simulink model "youBot_Arm"  (R2025a)
settings: Solver=ode15s  StartTime=0.0  StopTime=20  MaxStep=1e-2  RelTol=1e-3  AbsTol=1e-4
model workspace: external: MATLAB File youBot_DataFile.m (data not in the file)
undefined symbols (not defined in the file): Extr_Data_LinkHoles, Qt, sigbuilder_block, smiData, X, Y, YBT_Par, Z
libraries: sm_lib x193, nesl_utility x130, fl_lib x53, simulink x13, Parts_Lib x10, MyMath_lib x8, Motor_Lib x5, Contact_Forces_Lib x4, ee_lib x2, sdl_lib x2
(part 4 of 8)

== system youBot_Arm/Arm/Wrist/Wrist_1_RIGID ==
  ReferenceFrame : sm_lib/Frames and Transforms/Reference Frame
  Solid : sm_lib/Body Elements/File Solid  ExtGeomFileName=Wrist.step  UnitType=FromFile  ExtGeomFileUnits=m  StepReaderType=HEX  ExportConvexHullGeometry=off  InertiaType=Custom  BasedOnType=Density  Density=1000  DensityUnits=kg/m^3  Mass=smiData.Solid(9).mass  MassUnits=kg  CenterOfMass=smiData.Solid(9).CoM  CenterOfMassUnits=m  MomentsOfInertia=smiData.Solid(9).MoI  MomentsOfInertiaUnits=kg*m^2  ProductsOfInertia=smiData.Solid(9).PoI  ProductsOfInertiaUnits=kg*m^2  GraphicType=FromGeometry  MarkerShape=Sphere  MarkerSize=10  GraphicVisPropType=SimpleVisualProperties  GraphicDiffuseColor=smiData.Solid(9).color  GraphicOpacity=smiData.Solid(9).opacity  GraphicSpecularColor=[0.5 0.5 0.5 1.0]  GraphicAmbientColor=[0.15 0.15 0.15 1.0]  GraphicEmissiveColor=[0.0 0.0 0.0 1.0]  GraphicShininess=75  DoExposeReferenceFrame=on  SerializedFrames=<Frames/>
  Transform : sm_lib/Frames and Transforms/Rigid Transform  RotationMethod=ArbitraryAxis  FollAlignAxisA=+X  BaseAlignAxisA=+Y  FollAlignAxisB=+Y  BaseAlignAxisB=+Z  RotationStandardAxis=+Z  RotationAngle=smiData.RigidTransform(27).angle  RotationAngleUnits=rad  RotationArbitraryAxis=smiData.RigidTransform(27).axis  RotationSequenceAxes=FollowerAxes  RotationSequence=XYX  RotationSequenceAngles=[0 0 0]  RotationSequenceAnglesUnits=deg  RotationMatrix=[1 0 0; 0 1 0; 0 0 1]  Quaternion=[1 0 0 0]  TranslationMethod=Cartesian  TranslationCartesianOffset=smiData.RigidTransform(27).translation  TranslationCartesianOffsetUnits=m  TranslationStandardAxis=+Z  TranslationStandardOffset=0  TranslationStandardOffsetUnits=m  TranslationROffset=0  TranslationROffsetUnits=m  TranslationThetaOffset=0  TranslationThetaOffsetUnits=deg  TranslationZOffset=0  TranslationZOffsetUnits=m
  Transform1 : sm_lib/Frames and Transforms/Rigid Transform  RotationMethod=ArbitraryAxis  FollAlignAxisA=+X  BaseAlignAxisA=+Y  FollAlignAxisB=+Y  BaseAlignAxisB=+Z  RotationStandardAxis=+Z  RotationAngle=smiData.RigidTransform(30).angle  RotationAngleUnits=rad  RotationArbitraryAxis=smiData.RigidTransform(30).axis  RotationSequenceAxes=FollowerAxes  RotationSequence=XYX  RotationSequenceAngles=[0 0 0]  RotationSequenceAnglesUnits=deg  RotationMatrix=[1 0 0; 0 1 0; 0 0 1]  Quaternion=[1 0 0 0]  TranslationMethod=Cartesian  TranslationCartesianOffset=smiData.RigidTransform(30).translation  TranslationCartesianOffsetUnits=m  TranslationStandardAxis=+Z  TranslationStandardOffset=0  TranslationStandardOffsetUnits=m  TranslationROffset=0  TranslationROffsetUnits=m  TranslationThetaOffset=0  TranslationThetaOffsetUnits=deg  TranslationZOffset=0  TranslationZOffsetUnits=m
  F1 : PMIOPort  Side=Left
  F : PMIOPort  Port=2  Side=Right
  connections:
  Solid/RConn1 -- ReferenceFrame/RConn1 -- Transform/LConn1 -- Transform1/LConn1
  Transform/RConn1 -- F/RConn1
  Transform1/RConn1 -- F1/RConn1

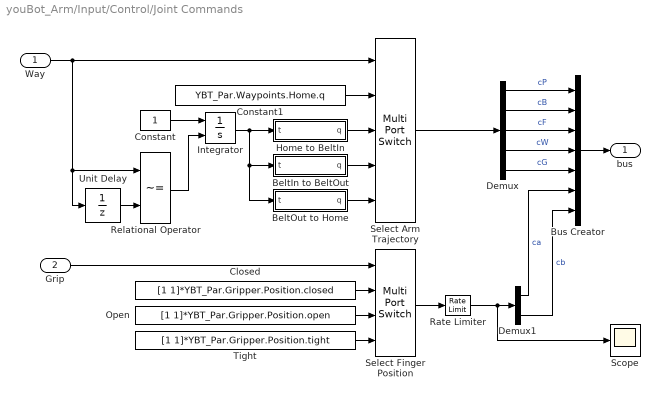
== system youBot_Arm/Input/Control/Joint Commands ==
  Way : Inport
  Grip : Inport  Port=2
  BeltIn to BeltOut : Subsystem
  BeltOut to Home : Subsystem
  Bus Creator : BusCreator  Inputs=7
  Closed : Constant  Value=[1 1]*YBT_Par.Gripper.Position.closed
  Constant : Constant  SampleTime=0
  Constant1 : Constant  Value=YBT_Par.Waypoints.Home.q
  Demux : Demux  Outputs=5
  Demux1 : Demux  Outputs=2
  Home to BeltIn : Subsystem
  Integrator : Integrator  ExternalReset=rising
  Open : Constant  Value=[1 1]*YBT_Par.Gripper.Position.open
  Rate Limiter : RateLimiter  RisingSlewLimit=YBT_Par.Finger_A.Motor.max_spd  FallingSlewLimit=-YBT_Par.Finger_A.Motor.max_spd  SampleTimeMode=inherited
  Relational Operator : RelationalOperator  Operator=~=  OutDataTypeStr=boolean  RndMeth=Simplest  InputSameDT=off
  Scope : Scope
      settings: ActiveDisplayYMinimum=-4.375  ActiveDisplayYMaximum=39.375
  Select Arm Trajectory : MultiPortSwitch  DataPortOrder=Zero-based contiguous  Inputs=4  zeroidx=on  SaturateOnIntegerOverflow=off  InputSameDT=off
  Select Finger Position : MultiPortSwitch  DataPortOrder=Zero-based contiguous  zeroidx=on  SaturateOnIntegerOverflow=off  InputSameDT=off
  Tight : Constant  Value=[1 1]*YBT_Par.Gripper.Position.tight
  Unit Delay : UnitDelay  SampleTime=1e-2  HasFrameUpgradeWarning=on
  bus : Outport  VectorParamsAs1DForOutWhenUnconnected=off
  wires:
  Bus Creator/1 -> bus/1
  Demux/5 -> Bus Creator/5  "cG"
  Demux/4 -> Bus Creator/4  "cW"
  Demux/3 -> Bus Creator/3  "cF"
  Demux/2 -> Bus Creator/2  "cB"
  Demux1/2 -> Bus Creator/7  "cb"
  Demux1/1 -> Bus Creator/6  "ca"
  Select Finger Position/1 -> Rate Limiter/1
  Grip/1 -> Select Finger Position/1
  Tight/1 -> Select Finger Position/4
  Open/1 -> Select Finger Position/3
  Closed/1 -> Select Finger Position/2
  Demux/1 -> Bus Creator/1  "cP"
  Integrator/1 -> BeltOut to Home/1(t), BeltIn to BeltOut/1(t), Home to BeltIn/1(t)
  Constant1/1 -> Select Arm Trajectory/2
  Relational Operator/1 -> Integrator/2
  Select Arm Trajectory/1 -> Demux/1
  Home to BeltIn/1(q) -> Select Arm Trajectory/3
  BeltIn to BeltOut/1(q) -> Select Arm Trajectory/4
  Unit Delay/1 -> Relational Operator/2
  Constant/1 -> Integrator/1
  Way/1 -> Select Arm Trajectory/1, Relational Operator/1, Unit Delay/1
  BeltOut to Home/1(q) -> Select Arm Trajectory/5
  Rate Limiter/1 -> Scope/1, Demux1/1

== system youBot_Arm/Input/Control/Logging ==
  S : Inport
  Bus Selector1 : BusSelector  Commented=on  OutputSignals=BeltIn.Box,BeltIn.LC,BeltOut.Box,BeltOut.LC
  Bus Selector2 : BusSelector  Commented=on  OutputSignals=Belts
  From Workspace : FromWorkspace  Commented=on  VariableName=chartInputs  OutDataTypeStr=Bus: Belts
  Scope : Scope  Commented=on  NumInputPorts=4
      settings: ActiveDisplayYMinimum=-0.125  ActiveDisplayYMaximum=1.125
  To Workspace : ToWorkspace  Commented=on  VariableName=chartInputs  SaveFormat=Timeseries  SampleTime=0.1
  wires:
  From Workspace/1 -> Bus Selector1/1
  Bus Selector1/2 -> Scope/2  "<LC>"
  Bus Selector1/3 -> Scope/3  "<Box>"
  Bus Selector1/4 -> Scope/4  "<LC>"
  Bus Selector1/1 -> Scope/1  "<Box>"
  Bus Selector2/1 -> To Workspace/1  "<Belts>"
  S/1 -> Bus Selector2/1

== system youBot_Arm/Input/Control Belt/Control Belt In ==
  BeltOut : Inport
  Sensor : Inport  Port=2
  Product : Product
  Scope : Scope  NumInputPorts=3
      settings: ActiveDisplayYMinimum=-0.125  ActiveDisplayYMaximum=1.125
  On : Outport  VectorParamsAs1DForOutWhenUnconnected=off
  wires:
  Sensor/1 -> Scope/3, Product/2
  Product/1 -> Scope/1, On/1  "vx"
  BeltOut/1 -> Scope/2, Product/1

== system youBot_Arm/Input/Control Belt/Control Belt Out ==
  BeltOut : Inport
  Sensor : Inport  Port=2
  Product : Product
  Scope : Scope  NumInputPorts=3
      settings: ActiveDisplayYMinimum=-0.125  ActiveDisplayYMaximum=1.125
  On : Outport  VectorParamsAs1DForOutWhenUnconnected=off
  wires:
  BeltOut/1 -> Product/1, Scope/2
  Product/1 -> On/1, Scope/1  "vx"
  Sensor/1 -> Product/2, Scope/3

== system youBot_Arm/Input/Control Belt/Robot Commands ==
  Bus Creator : BusCreator  Tag=Bus Creator  Inputs=7
  FromWs : FromWorkspace  Tag=STV FromWs  VariableName=tuvar
      SigBuilderData=|
      | common.afterFinalStr = 'Extrapolate'
      | common.sampleTime = 0
      | dataSet(1).timeRange = [0 10]
      | dataSet(1).name = 'All 35'
      | dataSet(2).timeRange = [0 20]
      | dataSet(2).name = 'Box 40 cm'
      | dataSet(3).timeRange = [0 20]
      | dataSet(3).name = 'Box 40 cm Flip'
      | dataSet(4).timeRange = [0 20]
      | dataSet(4).name = 'Box 40 cm upDown'
      | dataSet(5).timeRange = [0 3]
      | dataSet(5).name = 'Opt Flip Orig'
      | dataSet(6).timeRange = [0 4]
      | dataSet(6).name = 'Opt Flip Test'
      | dataSet(7).timeRange = [0 14]
      | dataSet(7).name = 'Test Pivot'
      | dataSet(8).timeRange = [0 14]
      | dataSet(8).name = 'Test Bicep'
      | dataSet(9).timeRange = [0 14]
      | dataSet(9).name = 'Test Forearm'
      | dataSet(10).timeRange = [0 14]
      | dataSet(10).name = 'Test Wrist'
      | sbobj.Groups(1).Name = 'All 35'
      | sbobj.Groups(1).Signals(1).Name = 'cP'
      | sbobj.Groups(1).Signals(1).XData = [0 2 4 6 8 10]
      | sbobj.Groups(1).Signals(1).YData = [0 0 35 35 0 0]
      | sbobj.Groups(1).Signals(2).Name = 'cB'
      | sbobj.Groups(1).Signals(2).XData = [0 2 4 6 8 10]
      | sbobj.Groups(1).Signals(2).YData = [0 0 35 35 0 0]
      | sbobj.Groups(1).Signals(3).Name = 'cF'
      | sbobj.Groups(1).Signals(3).XData = [0 2 4 6 8 10]
      | sbobj.Groups(1).Signals(3).YData = [0 0 35 35 0 0]
      | sbobj.Groups(1).Signals(4).Name = 'cW'
      | sbobj.Groups(1).Signals(4).XData = [0 2 4 6 8 10]
      | sbobj.Groups(1).Signals(4).YData = [0 0 35 35 0 0]
      | sbobj.Groups(1).Signals(5).Name = 'cG'
      | sbobj.Groups(1).Signals(5).XData = [0 2 4 6 8 10]
      | sbobj.Groups(1).Signals(5).YData = [0 0 35 35 0 0]
      | sbobj.Groups(1).Signals(6).Name = 'ca'
      | sbobj.Groups(1).Signals(6).XData = [0 2 4 6 8 10]
      | sbobj.Groups(1).Signals(6).YData = [0 0 35 35 0 0]
      | sbobj.Groups(1).Signals(7).Name = 'cb'
      | sbobj.Groups(1).Signals(7).XData = [0 2 4 6 8 10]
      | sbobj.Groups(1).Signals(7).YData = [0 0 35 35 0 0]
      | sbobj.Groups(2).Name = 'Box 40 cm'
      | sbobj.Groups(2).Signals(1).Name = 'cP'
      | sbobj.Groups(2).Signals(1).XData = [0 2 4 5.5 7 9 14 18 20]
      | sbobj.Groups(2).Signals(1).YData = [0 0 0 0 0 -90 -90 0 0]
      | sbobj.Groups(2).Signals(2).Name = 'cB'
      | sbobj.Groups(2).Signals(2).XData = [0 2 4 6 7 8 10 13 18 20]
      | sbobj.Groups(2).Signals(2).YData = [0 0 60 60 50 50 59 59 0 0]
      | sbobj.Groups(2).Signals(3).Name = 'cF'
      | sbobj.Groups(2).Signals(3).XData = [0 2 3 14 18 20]
      | sbobj.Groups(2).Signals(3).YData = [0 0 115 115 0 0]
      | sbobj.Groups(2).Signals(4).Name = 'cW'
      | sbobj.Groups(2).Signals(4).XData = [0 2 4 14 18 20]
      | sbobj.Groups(2).Signals(4).YData = [0 0 -85 -85 0 0]
      | sbobj.Groups(2).Signals(5).Name = 'cG'
      | sbobj.Groups(2).Signals(5).XData = [0 2 4 6 8 20]
      | sbobj.Groups(2).Signals(5).YData = [0 0 0 0 0 0]
      | sbobj.Groups(2).Signals(6).Name = 'ca'
      | sbobj.Groups(2).Signals(6).XData = [0 2 3 4.5 5 12 12.2 20]
      | sbobj.Groups(2).Signals(6).YData = [0 0 35 35 29 29 31 31]
      | sbobj.Groups(2).Signals(7).Name = 'cb'
      | sbobj.Groups(2).Signals(7).XData = [0 2 3 4.5 5 12 12.2 20]
      | sbobj.Groups(2).Signals(7).YData = [0 0 35 35 29 29 31 31]
      | sbobj.Groups(2).TimeRange = [0 20]
      | sbobj.Groups(3).Name = 'Box 40 cm Flip'
      | sbobj.Groups(3).Signals(1).Name = 'cP'
      | sbobj.Groups(3).Signals(1).XData = [0 2 4 5.5 6 10 16 18 20]
      | sbobj.Groups(3).Signals(1).YData = [0 0 0 0 0 90 90 0 0]
      | sbobj.Groups(3).Signals(2).Name = 'cB'
      | sbobj.Groups(3).Signals(2).XData = [0 2 4 5.5 10 14 18 20]
      | sbobj.Groups(3).Signals(2).YData = [0 0 60 60 -60 -60 0 0]
      | sbobj.Groups(3).Signals(3).Name = 'cF'
      | sbobj.Groups(3).Signals(3).XData = [0 2 3.5 5.5 10 14 18 20]
      | sbobj.Groups(3).Signals(3).YData = [0 0 115 115 -110 -110 0 0]
      | sbobj.Groups(3).Signals(4).Name = 'cW'
      | sbobj.Groups(3).Signals(4).XData = [0 2 3.5 5.5 10 14 18 20]
      | sbobj.Groups(3).Signals(4).YData = [0 0 -85 -85 79 79 0 0]
      | sbobj.Groups(3).Signals(5).Name = 'cG'
      | sbobj.Groups(3).Signals(5).XData = [0 2 4 6 8 20]
      | sbobj.Groups(3).Signals(5).YData = [0 0 0 0 0 0]
      | sbobj.Groups(3).Signals(6).Name = 'ca'
      | sbobj.Groups(3).Signals(6).XData = [0 2 2.5 4.5 5 11.5 12 20]
      | sbobj.Groups(3).Signals(6).YData = [0 0 35 35 29 29 31 31]
      | sbobj.Groups(3).Signals(7).Name = 'cb'
      | sbobj.Groups(3).Signals(7).XData = [0 2 2.5 4.5 5 11.5 12 20]
      | sbobj.Groups(3).Signals(7).YData = [0 0 35 35 29 29 31 31]
      | sbobj.Groups(3).TimeRange = [0 20]
      | sbobj.Groups(4).Name = 'Box 40 cm upDown'
      | sbobj.Groups(4).Signals(1).Name = 'cP'
      | sbobj.Groups(4).Signals(1).XData = [0 2 4 5.5 7 9 14 18 20]
      | sbobj.Groups(4).Signals(1).YData = [0 0 0 0 0 360 360 0 0]
      | sbobj.Groups(4).Signals(2).Name = 'cB'
      | sbobj.Groups(4).Signals(2).XData = [0 2 4 6 7 8 10 13 18 20]
      | sbobj.Groups(4).Signals(2).YData = [0 0 60 60 50 50 59 59 0 0]
      | sbobj.Groups(4).Signals(3).Name = 'cF'
      | sbobj.Groups(4).Signals(3).XData = [0 2 3 14 18 20]
      | sbobj.Groups(4).Signals(3).YData = [0 0 115 115 0 0]
      | sbobj.Groups(4).Signals(4).Name = 'cW'
      | sbobj.Groups(4).Signals(4).XData = [0 2 4 14 18 20]
      | sbobj.Groups(4).Signals(4).YData = [0 0 -85 -85 0 0]
      | sbobj.Groups(4).Signals(5).Name = 'cG'
      | sbobj.Groups(4).Signals(5).XData = [0 2 4 6 8 20]
      | sbobj.Groups(4).Signals(5).YData = [0 0 0 0 0 0]
      | sbobj.Groups(4).Signals(6).Name = 'ca'
      | sbobj.Groups(4).Signals(6).XData = [0 2 3 4.5 5 12 12.2 20]
      | sbobj.Groups(4).Signals(6).YData = [0 0 35 35 29 29 31 31]
      | sbobj.Groups(4).Signals(7).Name = 'cb'
      | sbobj.Groups(4).Signals(7).XData = [0 2 3 4.5 5 12 12.2 20]
      | sbobj.Groups(4).Signals(7).YData = [0 0 35 35 29 29 31 31]
      | sbobj.Groups(4).TimeRange = [0 20]
      | sbobj.Groups(5).Name = 'Opt Flip Orig'
      | sbobj.Groups(5).Signals(1).Name = 'cP'
      | sbobj.Groups(5).Signals(1).XData = [0 3]
      | sbobj.Groups(5).Signals(1).YData = [0 90]
      | sbobj.Groups(5).Signals(2).Name = 'cB'
      | sbobj.Groups(5).Signals(2).XData = [0 3]
      | sbobj.Groups(5).Signals(2).YData = [60 -60]
      | sbobj.Groups(5).Signals(3).Name = 'cF'
      | sbobj.Groups(5).Signals(3).XData = [0 3]
      | sbobj.Groups(5).Signals(3).YData = [115 -110]
      | sbobj.Groups(5).Signals(4).Name = 'cW'
      | sbobj.Groups(5).Signals(4).XData = [0 3]
      | sbobj.Groups(5).Signals(4).YData = [-85 79]
      | sbobj.Groups(5).Signals(5).Name = 'cG'
      | sbobj.Groups(5).Signals(5).XData = [0 2 3]
      | sbobj.Groups(5).Signals(5).YData = [0 0 0]
      | sbobj.Groups(5).Signals(6).Name = 'ca'
      | sbobj.Groups(5).Signals(6).XData = [0 3]
      | sbobj.Groups(5).Signals(6).YData = [0 0]
      | sbobj.Groups(5).Signals(7).Name = 'cb'
      | sbobj.Groups(5).Signals(7).XData = [0 3]
      | sbobj.Groups(5).Signals(7).YData = [0 0]
      | sbobj.Groups(5).TimeRange = [0 3]
      | sbobj.Groups(6).Name = 'Opt Flip Test'
      | sbobj.Groups(6).Signals(1).Name = 'cP'
      | sbobj.Groups(6).Signals(1).XData = [0 3 4]
      | sbobj.Groups(6).Signals(1).YData = [0 90 90]
      | sbobj.Groups(6).Signals(2).Name = 'cB'
      | sbobj.Groups(6).Signals(2).XData = [0 3 4]
      | sbobj.Groups(6).Signals(2).YData = [60 -60 -60]
      | sbobj.Groups(6).Signals(3).Name = 'cF'
      | sbobj.Groups(6).Signals(3).XData = [0 3 4]
      | sbobj.Groups(6).Signals(3).YData = [115 -110 -110]
      | sbobj.Groups(6).Signals(4).Name = 'cW'
      | sbobj.Groups(6).Signals(4).XData = [0 3 4]
      | sbobj.Groups(6).Signals(4).YData = [-85 79 79]
      | sbobj.Groups(6).Signals(5).Name = 'cG'
      | sbobj.Groups(6).Signals(5).XData = [0 2 4]
      | sbobj.Groups(6).Signals(5).YData = [0 0 0]
      | sbobj.Groups(6).Signals(6).Name = 'ca'
      | sbobj.Groups(6).Signals(6).XData = [0 4]
      | sbobj.Groups(6).Signals(6).YData = [0 0]
      | sbobj.Groups(6).Signals(7).Name = 'cb'
      | sbobj.Groups(6).Signals(7).XData = [0 4]
      | sbobj.Groups(6).Signals(7).YData = [0 0]
      | sbobj.Groups(6).TimeRange = [0 4]
      | sbobj.Groups(7).Name = 'Test Pivot'
      | sbobj.Groups(7).Signals(1).Name = 'cP'
      | sbobj.Groups(7).Signals(1).XData = [0 2 4 5 8.8 10 12 14]
      | sbobj.Groups(7).Signals(1).YData = [0 0 -169 -169 169 169 0 0]
      | sbobj.Groups(7).Signals(2).Name = 'cB'
      | sbobj.Groups(7).Signals(2).XData = [0 2 3 5 6.73 8 8.72 14]
      | sbobj.Groups(7).Signals(2).YData = [0 0 0 0 0 0 0 0]
      | sbobj.Groups(7).Signals(3).Name = 'cF'
      | sbobj.Groups(7).Signals(3).XData = [0 2 3 5.5 10 14]
      | sbobj.Groups(7).Signals(3).YData = [0 0 0 0 0 0]
      | sbobj.Groups(7).Signals(4).Name = 'cW'
      | sbobj.Groups(7).Signals(4).XData = [0 2 4 5.5 10 14]
      | sbobj.Groups(7).Signals(4).YData = [0 0 0 0 0 0]
      | sbobj.Groups(7).Signals(5).Name = 'cG'
      | sbobj.Groups(7).Signals(5).XData = [0 2 4 6 8 14]
      | sbobj.Groups(7).Signals(5).YData = [0 0 0 0 0 0]
      | sbobj.Groups(7).Signals(6).Name = 'ca'
      | sbobj.Groups(7).Signals(6).XData = [0 2 2.5 4.5 5 11.5 12 14]
      | sbobj.Groups(7).Signals(6).YData = [0 0 0 0 0 0 0 0]
      | sbobj.Groups(7).Signals(7).Name = 'cb'
      | sbobj.Groups(7).Signals(7).XData = [0 2 2.5 4.5 5 11.5 12 14]
      | sbobj.Groups(7).Signals(7).YData = [0 0 0 0 0 0 0 0]
      | sbobj.Groups(7).TimeRange = [0 14]
      | sbobj.Groups(8).Name = 'Test Bicep'
      | sbobj.Groups(8).Signals(1).Name = 'cP'
      | sbobj.Groups(8).Signals(1).XData = [0 2 4 5.5 6 10 14]
      | sbobj.Groups(8).Signals(1).YData = [0 0 0 0 0 0 0]
      | sbobj.Groups(8).Signals(2).Name = 'cB'
      | sbobj.Groups(8).Signals(2).XData = [0 2 3 5 7 9 10 14]
      | sbobj.Groups(8).Signals(2).YData = [0 0 90 90 -65 -65 0 0]
      | sbobj.Groups(8).Signals(3).Name = 'cF'
      | sbobj.Groups(8).Signals(3).XData = [0 2 3 5.5 10 14]
      | sbobj.Groups(8).Signals(3).YData = [0 0 0 0 0 0]
      | sbobj.Groups(8).Signals(4).Name = 'cW'
      | sbobj.Groups(8).Signals(4).XData = [0 2 4 5.5 10 14]
      | sbobj.Groups(8).Signals(4).YData = [0 0 0 0 0 0]
      | sbobj.Groups(8).Signals(5).Name = 'cG'
      | sbobj.Groups(8).Signals(5).XData = [0 2 4 6 8 14]
      | sbobj.Groups(8).Signals(5).YData = [0 0 0 0 0 0]
      | sbobj.Groups(8).Signals(6).Name = 'ca'
      | sbobj.Groups(8).Signals(6).XData = [0 2 2.5 4.5 5 11.5 12 14]
      | sbobj.Groups(8).Signals(6).YData = [0 0 0 0 0 0 0 0]
      | sbobj.Groups(8).Signals(7).Name = 'cb'
      | sbobj.Groups(8).Signals(7).XData = [0 2 2.5 4.5 5 11.5 12 14]
      | sbobj.Groups(8).Signals(7).YData = [0 0 0 0 0 0 0 0]
      | sbobj.Groups(8).TimeRange = [0 14]
      | sbobj.Groups(9).Name = 'Test Forearm'
      | sbobj.Groups(9).Signals(1).Name = 'cP'
      | sbobj.Groups(9).Signals(1).XData = [0 2 4 5 8.8 10 12 14]
      | sbobj.Groups(9).Signals(1).YData = [0 0 0 0 0 0 0 0]
      | sbobj.Groups(9).Signals(2).Name = 'cB'
      | sbobj.Groups(9).Signals(2).XData = [0 2 3 5 6.73 8 8.72 14]
      | sbobj.Groups(9).Signals(2).YData = [0 0 0 0 0 0 0 0]
      | sbobj.Groups(9).Signals(3).Name = 'cF'
      | sbobj.Groups(9).Signals(3).XData = [0 2 3.7 5 8.8 10 11.6 14]
      | sbobj.Groups(9).Signals(3).YData = [0 0 -151 -151 90 90 0 0]
      | sbobj.Groups(9).Signals(4).Name = 'cW'
      | sbobj.Groups(9).Signals(4).XData = [0 2 4 5.5 10 14]
      | sbobj.Groups(9).Signals(4).YData = [0 0 0 0 0 0]
      | sbobj.Groups(9).Signals(5).Name = 'cG'
      | sbobj.Groups(9).Signals(5).XData = [0 2 4 6 8 14]
      | sbobj.Groups(9).Signals(5).YData = [0 0 0 0 0 0]
      | sbobj.Groups(9).Signals(6).Name = 'ca'
      | sbobj.Groups(9).Signals(6).XData = [0 2 2.5 4.5 5 11.5 12 14]
      | sbobj.Groups(9).Signals(6).YData = [0 0 0 0 0 0 0 0]
      | sbobj.Groups(9).Signals(7).Name = 'cb'
      | sbobj.Groups(9).Signals(7).XData = [0 2 2.5 4.5 5 11.5 12 14]
      | sbobj.Groups(9).Signals(7).YData = [0 0 0 0 0 0 0 0]
      | sbobj.Groups(9).TimeRange = [0 14]
      | sbobj.Groups(10).Name = 'Test Wrist'
      | sbobj.Groups(10).Signals(1).Name = 'cP'
      | sbobj.Groups(10).Signals(1).XData = [0 2 4 5 8.8 10 12 14]
      | sbobj.Groups(10).Signals(1).YData = [0 0 0 0 0 0 0 0]
      | sbobj.Groups(10).Signals(2).Name = 'cB'
      | sbobj.Groups(10).Signals(2).XData = [0 2 3 5 6.73 8 8.72 14]
      | sbobj.Groups(10).Signals(2).YData = [0 0 0 0 0 0 0 0]
      | sbobj.Groups(10).Signals(3).Name = 'cF'
      | sbobj.Groups(10).Signals(3).XData = [0 2 3 4 6 8 9 14]
      | sbobj.Groups(10).Signals(3).YData = [0 0 0 0 0 0 0 0]
      | sbobj.Groups(10).Signals(4).Name = 'cW'
      | sbobj.Groups(10).Signals(4).XData = [0 2 3.14 5 7.3 9 10.14 14]
      | sbobj.Groups(10).Signals(4).YData = [0 0 -102 -102 102 102 0 0]
      | sbobj.Groups(10).Signals(5).Name = 'cG'
      | sbobj.Groups(10).Signals(5).XData = [0 2 4 6 8 14]
      | sbobj.Groups(10).Signals(5).YData = [0 0 0 0 0 0]
      | sbobj.Groups(10).Signals(6).Name = 'ca'
      | sbobj.Groups(10).Signals(6).XData = [0 2 2.5 4.5 5 11.5 12 14]
      | sbobj.Groups(10).Signals(6).YData = [0 0 0 0 0 0 0 0]
      | sbobj.Groups(10).Signals(7).Name = 'cb'
      | sbobj.Groups(10).Signals(7).XData = [0 2 2.5 4.5 5 11.5 12 14]
      | sbobj.Groups(10).Signals(7).YData = [0 0 0 0 0 0 0 0]
      | sbobj.Groups(10).TimeRange = [0 14]
  Subsystem : Subsystem
  Bus : Outport  VectorParamsAs1DForOutWhenUnconnected=off
  wires:
  Subsystem/7(cb) -> Bus Creator/7  "cb"
  Subsystem/6(ca) -> Bus Creator/6  "ca"
  Subsystem/5(cG) -> Bus Creator/5  "cG"
  Subsystem/4(cW) -> Bus Creator/4  "cW"
  Subsystem/3(cF) -> Bus Creator/3  "cF"
  Subsystem/2(cB) -> Bus Creator/2  "cB"
  Subsystem/1(cP) -> Bus Creator/1  "cP"
  Bus Creator/1 -> Bus/1
  FromWs/1 -> Subsystem/1(In1)

== system youBot_Arm/Input/Signals/Belt Commands ==
  Bus Creator : BusCreator  Tag=Bus Creator  Inputs=2
  FromWs : FromWorkspace  Tag=STV FromWs  VariableName=tuvar
      SigBuilderData=|
      | common.afterFinalStr = 'Extrapolate'
      | common.sampleTime = 0
      | dataSet(1).timeRange = [0 10]
      | dataSet(1).name = 'Locked'
      | dataSet(2).timeRange = [0 20]
      | dataSet(2).name = 'Move Box'
      | sbobj.Groups(1).Name = 'Locked'
      | sbobj.Groups(1).Signals(1).Name = 'Belt In On'
      | sbobj.Groups(1).Signals(1).XData = [0 10]
      | sbobj.Groups(1).Signals(1).YData = [0 0]
      | sbobj.Groups(1).Signals(2).Name = 'Belt Out On'
      | sbobj.Groups(1).Signals(2).XData = [0 10]
      | sbobj.Groups(1).Signals(2).YData = [0 0]
      | sbobj.Groups(2).Name = 'Move Box'
      | sbobj.Groups(2).Signals(1).Name = 'Belt In On'
      | sbobj.Groups(2).Signals(1).XData = [0 0.5 0.5 1 2.5 2.5 20]
      | sbobj.Groups(2).Signals(1).YData = [0 0 1 1 1 0 0]
      | sbobj.Groups(2).Signals(2).Name = 'Belt Out On'
      | sbobj.Groups(2).Signals(2).XData = [0 14 14 17 17 20]
      | sbobj.Groups(2).Signals(2).YData = [0 0 1 1 0 0]
      | sbobj.Groups(2).TimeRange = [0 20]
  Subsystem : Subsystem
  Bus : Outport  VectorParamsAs1DForOutWhenUnconnected=off
  wires:
  FromWs/1 -> Subsystem/1(In1)
  Subsystem/1(Belt In On) -> Bus Creator/1  "Belt In On"
  Subsystem/2(Belt Out On) -> Bus Creator/2  "Belt Out On"
  Bus Creator/1 -> Bus/1

== system youBot_Arm/Input/Signals/Robot Commands ==
  Bus Creator : BusCreator  Tag=Bus Creator  Inputs=7
  FromWs : FromWorkspace  Tag=STV FromWs  VariableName=tuvar  OutputAfterFinalValue=Holding final value
      SigBuilderData=|
      | common.afterFinalStr = 'Hold final value'
      | common.sampleTime = '0'
      | dataSet(1).timeRange = [0 20]
      | dataSet(1).name = 'Box 40 cm'
      | dataSet(2).timeRange = [0 20]
      | dataSet(2).name = 'Box 40 cm Flip'
      | dataSet(3).timeRange = [0 20]
      | dataSet(3).name = 'Box 40 cm upDown'
      | dataSet(4).timeRange = [0 3]
      | dataSet(4).name = 'Opt Flip Orig'
      | dataSet(5).timeRange = [0 4]
      | dataSet(5).name = 'Opt Flip Test'
      | dataSet(6).timeRange = [0 14]
      | dataSet(6).name = 'Test Pivot'
      | dataSet(7).timeRange = [0 7]
      | dataSet(7).name = 'Test Bicep'
      | dataSet(8).timeRange = [0 10.5]
      | dataSet(8).name = 'Test Forearm'
      | dataSet(9).timeRange = [0 8.5]
      | dataSet(9).name = 'Test Wrist'
      | dataSet(10).timeRange = [0 6]
      | dataSet(10).name = 'Test Max Torque'
      | dataSet(11).timeRange = [0 5]
      | dataSet(11).name = 'Test All 35'
      | sbobj.Groups(1).Name = 'Box 40 cm'
      | sbobj.Groups(1).Signals(1).Name = 'cP'
      | sbobj.Groups(1).Signals(1).XData = [0 2 4 5.5 7 9 14 18 20]
      | sbobj.Groups(1).Signals(1).YData = [0 0 0 0 0 -90 -90 0 0]
      | sbobj.Groups(1).Signals(2).Name = 'cB'
      | sbobj.Groups(1).Signals(2).XData = [0 2 4 6 7 8 10 13 18 20]
      | sbobj.Groups(1).Signals(2).YData = [0 0 60 60 50 50 59 59 0 0]
      | sbobj.Groups(1).Signals(3).Name = 'cF'
      | sbobj.Groups(1).Signals(3).XData = [0 2 3 14 18 20]
      | sbobj.Groups(1).Signals(3).YData = [0 0 115 115 0 0]
      | sbobj.Groups(1).Signals(4).Name = 'cW'
      | sbobj.Groups(1).Signals(4).XData = [0 2 4 14 18 20]
      | sbobj.Groups(1).Signals(4).YData = [0 0 -85 -85 0 0]
      | sbobj.Groups(1).Signals(5).Name = 'cG'
      | sbobj.Groups(1).Signals(5).XData = [0 2 4 6 8 20]
      | sbobj.Groups(1).Signals(5).YData = [0 0 0 0 0 0]
      | sbobj.Groups(1).Signals(6).Name = 'ca'
      | sbobj.Groups(1).Signals(6).XData = [0 2 3 4.5 5 12 12.2 20]
      | sbobj.Groups(1).Signals(6).YData = [0 0 35 35 29 29 31 31]
      | sbobj.Groups(1).Signals(7).Name = 'cb'
      | sbobj.Groups(1).Signals(7).XData = [0 2 3 4.5 5 12 12.2 20]
      | sbobj.Groups(1).Signals(7).YData = [0 0 35 35 29 29 31 31]
      | sbobj.Groups(1).TimeRange = [0 20]
      | sbobj.Groups(2).Name = 'Box 40 cm Flip'
      | sbobj.Groups(2).Signals(1).Name = 'cP'
      | sbobj.Groups(2).Signals(1).XData = [0 2 4 5.5 6 10 16 18 20]
      | sbobj.Groups(2).Signals(1).YData = [0 0 0 0 0 90 90 0 0]
      | sbobj.Groups(2).Signals(2).Name = 'cB'
      | sbobj.Groups(2).Signals(2).XData = [0 2 4 5.5 10 14 18 20]
      | sbobj.Groups(2).Signals(2).YData = [0 0 60 60 -60 -60 0 0]
      | sbobj.Groups(2).Signals(3).Name = 'cF'
      | sbobj.Groups(2).Signals(3).XData = [0 2 3.5 5.5 10 14 18 20]
      | sbobj.Groups(2).Signals(3).YData = [0 0 115 115 -110 -110 0 0]
      | sbobj.Groups(2).Signals(4).Name = 'cW'
      | sbobj.Groups(2).Signals(4).XData = [0 2 3.5 5.5 10 14 18 20]
      | sbobj.Groups(2).Signals(4).YData = [0 0 -85 -85 80 80 0 0]
      | sbobj.Groups(2).Signals(5).Name = 'cG'
      | sbobj.Groups(2).Signals(5).XData = [0 2 4 6 8 20]
      | sbobj.Groups(2).Signals(5).YData = [0 0 0 0 0 0]
      | sbobj.Groups(2).Signals(6).Name = 'ca'
      | sbobj.Groups(2).Signals(6).XData = [0 2 2.5 4.5 5 11.5 12 20]
      | sbobj.Groups(2).Signals(6).YData = [0 0 35 35 29 29 31 31]
      | sbobj.Groups(2).Signals(7).Name = 'cb'
      | sbobj.Groups(2).Signals(7).XData = [0 2 2.5 4.5 5 11.5 12 20]
      | sbobj.Groups(2).Signals(7).YData = [0 0 35 35 29 29 31 31]
      | sbobj.Groups(2).TimeRange = [0 20]
      | sbobj.Groups(3).Name = 'Box 40 cm upDown'
      | sbobj.Groups(3).Signals(1).Name = 'cP'
      | sbobj.Groups(3).Signals(1).XData = [0 2 4 5.5 7 9 14 18 20]
      | sbobj.Groups(3).Signals(1).YData = [0 0 0 0 0 360 360 0 0]
      | sbobj.Groups(3).Signals(2).Name = 'cB'
      | sbobj.Groups(3).Signals(2).XData = [0 2 4 6 7 8 10 13 18 20]
      | sbobj.Groups(3).Signals(2).YData = [0 0 60 60 50 50 59 59 0 0]
      | sbobj.Groups(3).Signals(3).Name = 'cF'
      | sbobj.Groups(3).Signals(3).XData = [0 2 3 14 18 20]
      | sbobj.Groups(3).Signals(3).YData = [0 0 115 115 0 0]
      | sbobj.Groups(3).Signals(4).Name = 'cW'
      | sbobj.Groups(3).Signals(4).XData = [0 2 4 14 18 20]
      | sbobj.Groups(3).Signals(4).YData = [0 0 -85 -85 0 0]
      | sbobj.Groups(3).Signals(5).Name = 'cG'
      | sbobj.Groups(3).Signals(5).XData = [0 2 4 6 8 20]
      | sbobj.Groups(3).Signals(5).YData = [0 0 0 0 0 0]
      | sbobj.Groups(3).Signals(6).Name = 'ca'
      | sbobj.Groups(3).Signals(6).XData = [0 2 3 4.5 5 12 12.2 20]
      | sbobj.Groups(3).Signals(6).YData = [0 0 35 35 29 29 31 31]
      | sbobj.Groups(3).Signals(7).Name = 'cb'
      | sbobj.Groups(3).Signals(7).XData = [0 2 3 4.5 5 12 12.2 20]
      | sbobj.Groups(3).Signals(7).YData = [0 0 35 35 29 29 31 31]
      | sbobj.Groups(3).TimeRange = [0 20]
      | sbobj.Groups(4).Name = 'Opt Flip Orig'
      | sbobj.Groups(4).Signals(1).Name = 'cP'
      | sbobj.Groups(4).Signals(1).XData = [0 3]
      | sbobj.Groups(4).Signals(1).YData = [0 90]
      | sbobj.Groups(4).Signals(2).Name = 'cB'
      | sbobj.Groups(4).Signals(2).XData = [0 3]
      | sbobj.Groups(4).Signals(2).YData = [60 -60]
      | sbobj.Groups(4).Signals(3).Name = 'cF'
      | sbobj.Groups(4).Signals(3).XData = [0 3]
      | sbobj.Groups(4).Signals(3).YData = [115 -110]
      | sbobj.Groups(4).Signals(4).Name = 'cW'
      | sbobj.Groups(4).Signals(4).XData = [0 3]
      | sbobj.Groups(4).Signals(4).YData = [-85 79]
      | sbobj.Groups(4).Signals(5).Name = 'cG'
      | sbobj.Groups(4).Signals(5).XData = [0 2 3]
      | sbobj.Groups(4).Signals(5).YData = [0 0 0]
      | sbobj.Groups(4).Signals(6).Name = 'ca'
      | sbobj.Groups(4).Signals(6).XData = [0 3]
      | sbobj.Groups(4).Signals(6).YData = [0 0]
      | sbobj.Groups(4).Signals(7).Name = 'cb'
      | sbobj.Groups(4).Signals(7).XData = [0 3]
      | sbobj.Groups(4).Signals(7).YData = [0 0]
      | sbobj.Groups(4).TimeRange = [0 3]
      | sbobj.Groups(5).Name = 'Opt Flip Test'
      | sbobj.Groups(5).Signals(1).Name = 'cP'
      | sbobj.Groups(5).Signals(1).XData = [0 3 4]
      | sbobj.Groups(5).Signals(1).YData = [0 90 90]
      | sbobj.Groups(5).Signals(2).Name = 'cB'
      | sbobj.Groups(5).Signals(2).XData = [0 3 4]
      | sbobj.Groups(5).Signals(2).YData = [60 -60 -60]
      | sbobj.Groups(5).Signals(3).Name = 'cF'
      | sbobj.Groups(5).Signals(3).XData = [0 3 4]
      | sbobj.Groups(5).Signals(3).YData = [115 -110 -110]
      | sbobj.Groups(5).Signals(4).Name = 'cW'
      | sbobj.Groups(5).Signals(4).XData = [0 3 4]
      | sbobj.Groups(5).Signals(4).YData = [-85 79 79]
      | sbobj.Groups(5).Signals(5).Name = 'cG'
      | sbobj.Groups(5).Signals(5).XData = [0 2 4]
      | sbobj.Groups(5).Signals(5).YData = [0 0 0]
      | sbobj.Groups(5).Signals(6).Name = 'ca'
      | sbobj.Groups(5).Signals(6).XData = [0 4]
      | sbobj.Groups(5).Signals(6).YData = [0 0]
      | sbobj.Groups(5).Signals(7).Name = 'cb'
      | sbobj.Groups(5).Signals(7).XData = [0 4]
      | sbobj.Groups(5).Signals(7).YData = [0 0]
      | sbobj.Groups(5).TimeRange = [0 4]
      | sbobj.Groups(6).Name = 'Test Pivot'
      | sbobj.Groups(6).Signals(1).Name = 'cP'
      | sbobj.Groups(6).Signals(1).XData = [0 2 4 5 8.8 10 12 14]
      | sbobj.Groups(6).Signals(1).YData = [0 0 -169 -169 169 169 0 0]
      | sbobj.Groups(6).Signals(2).Name = 'cB'
      | sbobj.Groups(6).Signals(2).XData = [0 2 3 5 6.73 8 8.72 14]
      | sbobj.Groups(6).Signals(2).YData = [0 0 0 0 0 0 0 0]
      | sbobj.Groups(6).Signals(3).Name = 'cF'
      | sbobj.Groups(6).Signals(3).XData = [0 2 3 5.5 10 14]
      | sbobj.Groups(6).Signals(3).YData = [0 0 0 0 0 0]
      | sbobj.Groups(6).Signals(4).Name = 'cW'
      | sbobj.Groups(6).Signals(4).XData = [0 2 4 5.5 10 14]
      | sbobj.Groups(6).Signals(4).YData = [0 0 0 0 0 0]
      | sbobj.Groups(6).Signals(5).Name = 'cG'
      | sbobj.Groups(6).Signals(5).XData = [0 2 4 6 8 14]
      | sbobj.Groups(6).Signals(5).YData = [0 0 0 0 0 0]
      | sbobj.Groups(6).Signals(6).Name = 'ca'
      | sbobj.Groups(6).Signals(6).XData = [0 14]
      | sbobj.Groups(6).Signals(6).YData = [29 29]
      | sbobj.Groups(6).Signals(7).Name = 'cb'
      | sbobj.Groups(6).Signals(7).XData = [0 14]
      | sbobj.Groups(6).Signals(7).YData = [29 29]
      | sbobj.Groups(6).TimeRange = [0 14]
      | sbobj.Groups(7).Name = 'Test Bicep'
      | sbobj.Groups(7).Signals(1).Name = 'cP'
      | sbobj.Groups(7).Signals(1).XData = [0 2 4 5.5 6 7]
      | sbobj.Groups(7).Signals(1).YData = [0 0 0 0 0 0]
      | sbobj.Groups(7).Signals(2).Name = 'cB'
      | sbobj.Groups(7).Signals(2).XData = [0 1 2 3 4.75 6 6.75 7]
      | sbobj.Groups(7).Signals(2).YData = [0 0 90 90 -65 -65 0 0]
      | sbobj.Groups(7).Signals(3).Name = 'cF'
      | sbobj.Groups(7).Signals(3).XData = [0 2 3 5.5 7]
      | sbobj.Groups(7).Signals(3).YData = [0 0 0 0 0]
      | sbobj.Groups(7).Signals(4).Name = 'cW'
      | sbobj.Groups(7).Signals(4).XData = [0 2 4 5.5 7]
      | sbobj.Groups(7).Signals(4).YData = [0 0 0 0 0]
      | sbobj.Groups(7).Signals(5).Name = 'cG'
      | sbobj.Groups(7).Signals(5).XData = [0 2 4 6 7]
      | sbobj.Groups(7).Signals(5).YData = [0 0 0 0 0]
      | sbobj.Groups(7).Signals(6).Name = 'ca'
      | sbobj.Groups(7).Signals(6).XData = [0 7]
      | sbobj.Groups(7).Signals(6).YData = [29 29]
      | sbobj.Groups(7).Signals(7).Name = 'cb'
      | sbobj.Groups(7).Signals(7).XData = [0 7]
      | sbobj.Groups(7).Signals(7).YData = [29 29]
      | sbobj.Groups(7).TimeRange = [0 7]
      | sbobj.Groups(8).Name = 'Test Forearm'
      | sbobj.Groups(8).Signals(1).Name = 'cP'
      | sbobj.Groups(8).Signals(1).XData = [0 2 4 5 8.8 10 10.5]
      | sbobj.Groups(8).Signals(1).YData = [0 0 0 0 0 0 0]
      | sbobj.Groups(8).Signals(2).Name = 'cB'
      | sbobj.Groups(8).Signals(2).XData = [0 2 3 5 6.73 8 8.72 10.5]
      | sbobj.Groups(8).Signals(2).YData = [0 0 0 0 0 0 0 0]
      | sbobj.Groups(8).Signals(3).Name = 'cF'
      | sbobj.Groups(8).Signals(3).XData = [0 1 2.7 4 7.8 9 10 10.5]
      | sbobj.Groups(8).Signals(3).YData = [0 0 -151 -151 90 90 0 0]
      | sbobj.Groups(8).Signals(4).Name = 'cW'
      | sbobj.Groups(8).Signals(4).XData = [0 2 4 5.5 10 10.5]
      | sbobj.Groups(8).Signals(4).YData = [0 0 0 0 0 0]
      | sbobj.Groups(8).Signals(5).Name = 'cG'
      | sbobj.Groups(8).Signals(5).XData = [0 2 4 6 8 10.5]
      | sbobj.Groups(8).Signals(5).YData = [0 0 0 0 0 0]
      | sbobj.Groups(8).Signals(6).Name = 'ca'
      | sbobj.Groups(8).Signals(6).XData = [0 10.5]
      | sbobj.Groups(8).Signals(6).YData = [29 29]
      | sbobj.Groups(8).Signals(7).Name = 'cb'
      | sbobj.Groups(8).Signals(7).XData = [0 10.5]
      | sbobj.Groups(8).Signals(7).YData = [29 29]
      | sbobj.Groups(8).TimeRange = [0 10.5]
      | sbobj.Groups(9).Name = 'Test Wrist'
      | sbobj.Groups(9).Signals(1).Name = 'cP'
      | sbobj.Groups(9).Signals(1).XData = [0 2 4 5 8.5]
      | sbobj.Groups(9).Signals(1).YData = [0 0 0 0 0]
      | sbobj.Groups(9).Signals(2).Name = 'cB'
      | sbobj.Groups(9).Signals(2).XData = [0 2 3 5 6.73 8 8.5]
      | sbobj.Groups(9).Signals(2).YData = [0 0 0 0 0 0 0]
      | sbobj.Groups(9).Signals(3).Name = 'cF'
      | sbobj.Groups(9).Signals(3).XData = [0 8.5]
      | sbobj.Groups(9).Signals(3).YData = [90 90]
      | sbobj.Groups(9).Signals(4).Name = 'cW'
      | sbobj.Groups(9).Signals(4).XData = [0 1 2.14 3 5.3 7 8.14 8.5]
      | sbobj.Groups(9).Signals(4).YData = [0 0 -102 -102 102 102 0 0]
      | sbobj.Groups(9).Signals(5).Name = 'cG'
      | sbobj.Groups(9).Signals(5).XData = [0 2 4 6 8 8.5]
      | sbobj.Groups(9).Signals(5).YData = [0 0 0 0 0 0]
      | sbobj.Groups(9).Signals(6).Name = 'ca'
      | sbobj.Groups(9).Signals(6).XData = [0 8.5]
      | sbobj.Groups(9).Signals(6).YData = [29 29]
      | sbobj.Groups(9).Signals(7).Name = 'cb'
      | sbobj.Groups(9).Signals(7).XData = [0 8.5]
      | sbobj.Groups(9).Signals(7).YData = [29 29]
      | sbobj.Groups(9).TimeRange = [0 8.5]
      | sbobj.Groups(10).Name = 'Test Max Torque'
      | sbobj.Groups(10).Signals(1).Name = 'cP'
      | sbobj.Groups(10).Signals(1).XData = [0 2 4 5 6]
      | sbobj.Groups(10).Signals(1).YData = [0 0 0 0 0]
      | sbobj.Groups(10).Signals(2).Name = 'cB'
      | sbobj.Groups(10).Signals(2).XData = [0 1 2 3.5 4 5 5.5 6]
      | sbobj.Groups(10).Signals(2).YData = [0 0 90 90 45 45 0 0]
      | sbobj.Groups(10).Signals(3).Name = 'cF'
      | sbobj.Groups(10).Signals(3).XData = [0 1 2 3 4 5 5.5 6]
      | sbobj.Groups(10).Signals(3).YData = [0 0 45 45 -45 -45 0 0]
      | sbobj.Groups(10).Signals(4).Name = 'cW'
      | sbobj.Groups(10).Signals(4).XData = [0 1 2 3 4 5 5.5 6]
      | sbobj.Groups(10).Signals(4).YData = [0 0 45 45 -45 -45 0 0]
      | sbobj.Groups(10).Signals(5).Name = 'cG'
      | sbobj.Groups(10).Signals(5).XData = [0 2 4 6]
      | sbobj.Groups(10).Signals(5).YData = [0 0 0 0]
      | sbobj.Groups(10).Signals(6).Name = 'ca'
      | sbobj.Groups(10).Signals(6).XData = [0 6]
      | sbobj.Groups(10).Signals(6).YData = [29 29]
      | sbobj.Groups(10).Signals(7).Name = 'cb'
      | sbobj.Groups(10).Signals(7).XData = [0 6]
      | sbobj.Groups(10).Signals(7).YData = [29 29]
      | sbobj.Groups(10).TimeRange = [0 6]
      | sbobj.Groups(11).Name = 'Test All 35'
      | sbobj.Groups(11).Signals(1).Name = 'cP'
      | sbobj.Groups(11).Signals(1).XData = [0 1 2 3 4 5]
      | sbobj.Groups(11).Signals(1).YData = [0 0 35 35 0 0]
      | sbobj.Groups(11).Signals(2).Name = 'cB'
      | sbobj.Groups(11).Signals(2).XData = [0 1 2 3 4 5]
      | sbobj.Groups(11).Signals(2).YData = [0 0 35 35 0 0]
      | sbobj.Groups(11).Signals(3).Name = 'cF'
      | sbobj.Groups(11).Signals(3).XData = [0 1 2 3 4 5]
      | sbobj.Groups(11).Signals(3).YData = [0 0 35 35 0 0]
      | sbobj.Groups(11).Signals(4).Name = 'cW'
      | sbobj.Groups(11).Signals(4).XData = [0 1 2 3 4 5]
      | sbobj.Groups(11).Signals(4).YData = [0 0 35 35 0 0]
      | sbobj.Groups(11).Signals(5).Name = 'cG'
      | sbobj.Groups(11).Signals(5).XData = [0 1 2 3 4 5]
      | sbobj.Groups(11).Signals(5).YData = [0 0 35 35 0 0]
      | sbobj.Groups(11).Signals(6).Name = 'ca'
      | sbobj.Groups(11).Signals(6).XData = [0 1 2 3 4 5]
      | sbobj.Groups(11).Signals(6).YData = [0 0 35 35 0 0]
      | sbobj.Groups(11).Signals(7).Name = 'cb'
      | sbobj.Groups(11).Signals(7).XData = [0 1 2 3 4 5]
      | sbobj.Groups(11).Signals(7).YData = [0 0 35 35 0 0]
      | sbobj.Groups(11).TimeRange = [0 5]
  Subsystem : Subsystem
  Bus : Outport  VectorParamsAs1DForOutWhenUnconnected=off
  wires:
  FromWs/1 -> Subsystem/1(In1)
  Bus Creator/1 -> Bus/1
  Subsystem/1(cP) -> Bus Creator/1  "cP"
  Subsystem/2(cB) -> Bus Creator/2  "cB"
  Subsystem/3(cF) -> Bus Creator/3  "cF"
  Subsystem/4(cW) -> Bus Creator/4  "cW"
  Subsystem/5(cG) -> Bus Creator/5  "cG"
  Subsystem/6(ca) -> Bus Creator/6  "ca"
  Subsystem/7(cb) -> Bus Creator/7  "cb"

== system youBot_Arm/Scopes/Logging/Log Constraint Forces ==
  In1 : Inport
  Bus Selector2 : BusSelector  OutputSignals=Arm.P.fc,Arm.B.fc,Arm.F.fc,Arm.W.fc,Arm.G.fc,Arm.a.fc,Arm.b.fc
  Mux2 : Mux  Inputs=7
  Scope : Scope  NumInputPorts=7
      settings: ActiveDisplayYMinimum=-30.20152  ActiveDisplayYMaximum=92.15057
  Out1 : Outport  VectorParamsAs1DForOutWhenUnconnected=off
  wires:
  Bus Selector2/1 -> Scope/1, Mux2/1  "<fc>"
  Bus Selector2/4 -> Scope/4, Mux2/4  "<fc>"
  Bus Selector2/2 -> Scope/2, Mux2/2  "<fc>"
  Bus Selector2/6 -> Scope/6, Mux2/6  "<fc>"
  Bus Selector2/7 -> Scope/7, Mux2/7  "<fc>"
  Bus Selector2/3 -> Scope/3, Mux2/3  "<fc>"
  Mux2/1 -> Out1/1
  Bus Selector2/5 -> Scope/5, Mux2/5  "<fc>"
  In1/1 -> Bus Selector2/1

== system youBot_Arm/Scopes/Logging/Log Joint Angles ==
  In1 : Inport
  Bus Selector2 : BusSelector  OutputSignals=Arm.P.q,Arm.B.q,Arm.F.q,Arm.W.q,Arm.G.q,Arm.a.p,Arm.b.p
  Mux2 : Mux  Inputs=7
  Out1 : Outport  VectorParamsAs1DForOutWhenUnconnected=off
  wires:
  In1/1 -> Bus Selector2/1
  Bus Selector2/4 -> Mux2/4  "<q>"
  Mux2/1 -> Out1/1
  Bus Selector2/2 -> Mux2/2  "<q>"
  Bus Selector2/7 -> Mux2/7  "<p>"
  Bus Selector2/6 -> Mux2/6  "<p>"
  Bus Selector2/3 -> Mux2/3  "<q>"
  Bus Selector2/5 -> Mux2/5  "<q>"
  Bus Selector2/1 -> Mux2/1  "<q>"

== system youBot_Arm/Scopes/Logging/Log Torques ==
  In1 : Inport
  Bus Selector2 : BusSelector  OutputSignals=Arm.P.t,Arm.B.t,Arm.F.t,Arm.W.t,Arm.G.t,Arm.a.f,Arm.b.f
  Mux2 : Mux  Inputs=7
  Out1 : Outport  VectorParamsAs1DForOutWhenUnconnected=off
  wires:
  Bus Selector2/1 -> Mux2/1  "<t>"
  Bus Selector2/5 -> Mux2/5  "<t>"
  Bus Selector2/3 -> Mux2/3  "<t>"
  Bus Selector2/6 -> Mux2/6  "<f>"
  Bus Selector2/7 -> Mux2/7  "<f>"
  Bus Selector2/2 -> Mux2/2  "<t>"
  Mux2/1 -> Out1/1
  Bus Selector2/4 -> Mux2/4  "<t>"
  In1/1 -> Bus Selector2/1

== system youBot_Arm/Arm/Actuation/Motion/Meas B ==
  Abs : Abs  ZeroCross=off  SaturateOnIntegerOverflow=off
  Bus Creator : BusCreator  Inputs=5
  Gain : Gain  Gain=YBT_Par.Bicep.Motor.K/YBT_Par.Bicep.Motor.gr
  PS-Simulink Converter : nesl_utility/PS-Simulink Converter  PhysicalDomain=network_engine_domain  SubClassName=ps_output  LeftPortType=input  RightPortType=output  PseudoPeriodic=off  Frequencies=[]  VectorFormat=1-D array  Unit=rad  AffineConversion=off
  PS-Simulink Converter1 : nesl_utility/PS-Simulink Converter  PhysicalDomain=network_engine_domain  SubClassName=ps_output  LeftPortType=input  RightPortType=output  PseudoPeriodic=off  Frequencies=[]  VectorFormat=1-D array  Unit=1  AffineConversion=off
  PS-Simulink Converter7 : nesl_utility/PS-Simulink Converter  PhysicalDomain=network_engine_domain  SubClassName=ps_output  LeftPortType=input  RightPortType=output  PseudoPeriodic=off  Frequencies=[]  VectorFormat=1-D array  Unit=rad/s  AffineConversion=off
  PS-Simulink Converter8 : nesl_utility/PS-Simulink Converter  PhysicalDomain=network_engine_domain  SubClassName=ps_output  LeftPortType=input  RightPortType=output  PseudoPeriodic=off  Frequencies=[]  VectorFormat=1-D array  Unit=N*m  AffineConversion=off
  q : PMIOPort  Side=Left
  w : PMIOPort  Port=2  Side=Left
  t : PMIOPort  Port=3  Side=Left
  fc : PMIOPort  Port=4  Side=Left
  B : Outport  VectorParamsAs1DForOutWhenUnconnected=off
  wires:
  PS-Simulink Converter/1 -> Bus Creator/1  "q"
  PS-Simulink Converter7/1 -> Bus Creator/2  "w"
  Bus Creator/1 -> B/1  "B"
  PS-Simulink Converter8/1 -> Gain/1, Bus Creator/3  "t"
  Abs/1 -> Bus Creator/4  "i"
  Gain/1 -> Abs/1
  PS-Simulink Converter1/1 -> Bus Creator/5  "fc"
  connections:
  PS-Simulink Converter/LConn1 -- q/RConn1
  PS-Simulink Converter7/LConn1 -- w/RConn1
  PS-Simulink Converter8/LConn1 -- t/RConn1
  PS-Simulink Converter1/LConn1 -- fc/RConn1

== system youBot_Arm/Arm/Actuation/Motion/Meas F ==
  Abs : Abs  ZeroCross=off  SaturateOnIntegerOverflow=off
  Bus Creator : BusCreator  Inputs=5
  Gain : Gain  Gain=YBT_Par.Forearm.Motor.K/YBT_Par.Forearm.Motor.gr
  PS-Simulink Converter : nesl_utility/PS-Simulink Converter  PhysicalDomain=network_engine_domain  SubClassName=ps_output  LeftPortType=input  RightPortType=output  PseudoPeriodic=off  Frequencies=[]  VectorFormat=1-D array  Unit=rad  AffineConversion=off
  PS-Simulink Converter1 : nesl_utility/PS-Simulink Converter  PhysicalDomain=network_engine_domain  SubClassName=ps_output  LeftPortType=input  RightPortType=output  PseudoPeriodic=off  Frequencies=[]  VectorFormat=1-D array  Unit=1  AffineConversion=off
  PS-Simulink Converter7 : nesl_utility/PS-Simulink Converter  PhysicalDomain=network_engine_domain  SubClassName=ps_output  LeftPortType=input  RightPortType=output  PseudoPeriodic=off  Frequencies=[]  VectorFormat=1-D array  Unit=rad/s  AffineConversion=off
  PS-Simulink Converter8 : nesl_utility/PS-Simulink Converter  PhysicalDomain=network_engine_domain  SubClassName=ps_output  LeftPortType=input  RightPortType=output  PseudoPeriodic=off  Frequencies=[]  VectorFormat=1-D array  Unit=N*m  AffineConversion=off
  q : PMIOPort  Side=Left
  w : PMIOPort  Port=2  Side=Left
  t : PMIOPort  Port=3  Side=Left
  fc : PMIOPort  Port=4  Side=Left
  F : Outport  VectorParamsAs1DForOutWhenUnconnected=off
  wires:
  Bus Creator/1 -> F/1  "F"
  PS-Simulink Converter7/1 -> Bus Creator/2  "w"
  PS-Simulink Converter/1 -> Bus Creator/1  "q"
  PS-Simulink Converter8/1 -> Gain/1, Bus Creator/3  "t"
  Abs/1 -> Bus Creator/4  "i"
  Gain/1 -> Abs/1
  PS-Simulink Converter1/1 -> Bus Creator/5  "fc"
  connections:
  PS-Simulink Converter8/LConn1 -- t/RConn1
  PS-Simulink Converter7/LConn1 -- w/RConn1
  PS-Simulink Converter/LConn1 -- q/RConn1
  PS-Simulink Converter1/LConn1 -- fc/RConn1

== system youBot_Arm/Arm/Actuation/Motion/Meas G ==
  Abs : Abs  ZeroCross=off  SaturateOnIntegerOverflow=off
  Bus Creator : BusCreator  Inputs=5
  Gain : Gain  Gain=YBT_Par.Gripper.Motor.K/YBT_Par.Gripper.Motor.gr
  PS-Simulink Converter : nesl_utility/PS-Simulink Converter  PhysicalDomain=network_engine_domain  SubClassName=ps_output  LeftPortType=input  RightPortType=output  PseudoPeriodic=off  Frequencies=[]  VectorFormat=1-D array  Unit=rad  AffineConversion=off
  PS-Simulink Converter1 : nesl_utility/PS-Simulink Converter  PhysicalDomain=network_engine_domain  SubClassName=ps_output  LeftPortType=input  RightPortType=output  PseudoPeriodic=off  Frequencies=[]  VectorFormat=1-D array  Unit=1  AffineConversion=off
  PS-Simulink Converter7 : nesl_utility/PS-Simulink Converter  PhysicalDomain=network_engine_domain  SubClassName=ps_output  LeftPortType=input  RightPortType=output  PseudoPeriodic=off  Frequencies=[]  VectorFormat=1-D array  Unit=rad/s  AffineConversion=off
  PS-Simulink Converter8 : nesl_utility/PS-Simulink Converter  PhysicalDomain=network_engine_domain  SubClassName=ps_output  LeftPortType=input  RightPortType=output  PseudoPeriodic=off  Frequencies=[]  VectorFormat=1-D array  Unit=N*m  AffineConversion=off
  q : PMIOPort  Side=Left
  w : PMIOPort  Port=2  Side=Left
  t : PMIOPort  Port=3  Side=Left
  fc : PMIOPort  Port=4  Side=Left
  G : Outport  VectorParamsAs1DForOutWhenUnconnected=off
  wires:
  PS-Simulink Converter/1 -> Bus Creator/1  "q"
  PS-Simulink Converter7/1 -> Bus Creator/2  "w"
  Bus Creator/1 -> G/1  "G"
  PS-Simulink Converter8/1 -> Gain/1, Bus Creator/3  "t"
  Abs/1 -> Bus Creator/4  "i"
  Gain/1 -> Abs/1
  PS-Simulink Converter1/1 -> Bus Creator/5  "fc"
  connections:
  PS-Simulink Converter/LConn1 -- q/RConn1
  PS-Simulink Converter7/LConn1 -- w/RConn1
  PS-Simulink Converter8/LConn1 -- t/RConn1
  PS-Simulink Converter1/LConn1 -- fc/RConn1

== system youBot_Arm/Arm/Actuation/Motion/Meas P ==
  Abs : Abs  ZeroCross=off  SaturateOnIntegerOverflow=off
  Bus Creator : BusCreator  Inputs=5
  Gain : Gain  Gain=YBT_Par.Pivot.Motor.K/YBT_Par.Pivot.Motor.gr
  PS-Simulink Converter : nesl_utility/PS-Simulink Converter  PhysicalDomain=network_engine_domain  SubClassName=ps_output  LeftPortType=input  RightPortType=output  PseudoPeriodic=off  Frequencies=[]  VectorFormat=1-D array  Unit=rad  AffineConversion=off
  PS-Simulink Converter1 : nesl_utility/PS-Simulink Converter  PhysicalDomain=network_engine_domain  SubClassName=ps_output  LeftPortType=input  RightPortType=output  PseudoPeriodic=off  Frequencies=[]  VectorFormat=1-D array  Unit=1  AffineConversion=off
  PS-Simulink Converter7 : nesl_utility/PS-Simulink Converter  PhysicalDomain=network_engine_domain  SubClassName=ps_output  LeftPortType=input  RightPortType=output  PseudoPeriodic=off  Frequencies=[]  VectorFormat=1-D array  Unit=rad/s  AffineConversion=off
  PS-Simulink Converter8 : nesl_utility/PS-Simulink Converter  PhysicalDomain=network_engine_domain  SubClassName=ps_output  LeftPortType=input  RightPortType=output  PseudoPeriodic=off  Frequencies=[]  VectorFormat=1-D array  Unit=N*m  AffineConversion=off
  q : PMIOPort  Side=Left
  w : PMIOPort  Port=2  Side=Left
  t : PMIOPort  Port=3  Side=Left
  fc : PMIOPort  Port=4  Side=Left
  P : Outport  VectorParamsAs1DForOutWhenUnconnected=off
  wires:
  PS-Simulink Converter/1 -> Bus Creator/1  "q"
  PS-Simulink Converter7/1 -> Bus Creator/2  "w"
  PS-Simulink Converter8/1 -> Gain/1, Bus Creator/3  "t"
  Bus Creator/1 -> P/1  "P"
  Abs/1 -> Bus Creator/4  "i"
  Gain/1 -> Abs/1
  PS-Simulink Converter1/1 -> Bus Creator/5  "fc"
  connections:
  PS-Simulink Converter/LConn1 -- q/RConn1
  PS-Simulink Converter7/LConn1 -- w/RConn1
  PS-Simulink Converter8/LConn1 -- t/RConn1
  PS-Simulink Converter1/LConn1 -- fc/RConn1

== system youBot_Arm/Arm/Actuation/Motion/Meas W ==
  Abs : Abs  ZeroCross=off  SaturateOnIntegerOverflow=off
  Bus Creator : BusCreator  Inputs=5
  Gain : Gain  Gain=YBT_Par.Wrist.Motor.K/YBT_Par.Wrist.Motor.gr
  PS-Simulink Converter : nesl_utility/PS-Simulink Converter  PhysicalDomain=network_engine_domain  SubClassName=ps_output  LeftPortType=input  RightPortType=output  PseudoPeriodic=off  Frequencies=[]  VectorFormat=1-D array  Unit=rad  AffineConversion=off
  PS-Simulink Converter1 : nesl_utility/PS-Simulink Converter  PhysicalDomain=network_engine_domain  SubClassName=ps_output  LeftPortType=input  RightPortType=output  PseudoPeriodic=off  Frequencies=[]  VectorFormat=1-D array  Unit=1  AffineConversion=off
  PS-Simulink Converter7 : nesl_utility/PS-Simulink Converter  PhysicalDomain=network_engine_domain  SubClassName=ps_output  LeftPortType=input  RightPortType=output  PseudoPeriodic=off  Frequencies=[]  VectorFormat=1-D array  Unit=rad/s  AffineConversion=off
  PS-Simulink Converter8 : nesl_utility/PS-Simulink Converter  PhysicalDomain=network_engine_domain  SubClassName=ps_output  LeftPortType=input  RightPortType=output  PseudoPeriodic=off  Frequencies=[]  VectorFormat=1-D array  Unit=N*m  AffineConversion=off
  q : PMIOPort  Side=Left
  w : PMIOPort  Port=2  Side=Left
  t : PMIOPort  Port=3  Side=Left
  fc : PMIOPort  Port=4  Side=Left
  W : Outport  VectorParamsAs1DForOutWhenUnconnected=off
  wires:
  Bus Creator/1 -> W/1  "W"
  PS-Simulink Converter7/1 -> Bus Creator/2  "w"
  PS-Simulink Converter/1 -> Bus Creator/1  "q"
  PS-Simulink Converter8/1 -> Gain/1, Bus Creator/3  "t"
  Abs/1 -> Bus Creator/4  "i"
  Gain/1 -> Abs/1
  PS-Simulink Converter1/1 -> Bus Creator/5  "fc"
  connections:
  PS-Simulink Converter8/LConn1 -- t/RConn1
  PS-Simulink Converter7/LConn1 -- w/RConn1
  PS-Simulink Converter/LConn1 -- q/RConn1
  PS-Simulink Converter1/LConn1 -- fc/RConn1

== system youBot_Arm/Arm/Actuation/Motion/Meas a ==
  Abs : Abs  ZeroCross=off  SaturateOnIntegerOverflow=off
  Bus Creator : BusCreator  Inputs=5
  Gain : Gain  Gain=YBT_Par.Finger_A.Motor.K/YBT_Par.Finger_A.Motor.gr
  PS-Simulink Converter : nesl_utility/PS-Simulink Converter  PhysicalDomain=network_engine_domain  SubClassName=ps_output  LeftPortType=input  RightPortType=output  PseudoPeriodic=off  Frequencies=[]  VectorFormat=1-D array  Unit=mm  AffineConversion=off
  PS-Simulink Converter1 : nesl_utility/PS-Simulink Converter  PhysicalDomain=network_engine_domain  SubClassName=ps_output  LeftPortType=input  RightPortType=output  PseudoPeriodic=off  Frequencies=[]  VectorFormat=1-D array  Unit=1  AffineConversion=off
  PS-Simulink Converter7 : nesl_utility/PS-Simulink Converter  PhysicalDomain=network_engine_domain  SubClassName=ps_output  LeftPortType=input  RightPortType=output  PseudoPeriodic=off  Frequencies=[]  VectorFormat=1-D array  Unit=mm/s  AffineConversion=off
  PS-Simulink Converter8 : nesl_utility/PS-Simulink Converter  PhysicalDomain=network_engine_domain  SubClassName=ps_output  LeftPortType=input  RightPortType=output  PseudoPeriodic=off  Frequencies=[]  VectorFormat=1-D array  Unit=N  AffineConversion=off
  p : PMIOPort  Side=Left
  v : PMIOPort  Port=2  Side=Left
  f : PMIOPort  Port=3  Side=Left
  fc : PMIOPort  Port=4  Side=Left
  a : Outport  VectorParamsAs1DForOutWhenUnconnected=off
  wires:
  PS-Simulink Converter/1 -> Bus Creator/1  "p"
  PS-Simulink Converter7/1 -> Bus Creator/2  "v"
  Bus Creator/1 -> a/1  "a"
  PS-Simulink Converter8/1 -> Gain/1, Bus Creator/3  "f"
  Abs/1 -> Bus Creator/4  "i"
  Gain/1 -> Abs/1
  PS-Simulink Converter1/1 -> Bus Creator/5  "fc"
  connections:
  PS-Simulink Converter/LConn1 -- p/RConn1
  PS-Simulink Converter7/LConn1 -- v/RConn1
  PS-Simulink Converter8/LConn1 -- f/RConn1
  PS-Simulink Converter1/LConn1 -- fc/RConn1

== system youBot_Arm/Arm/Actuation/Motion/Meas b ==
  Abs : Abs  ZeroCross=off  SaturateOnIntegerOverflow=off
  Bus Creator : BusCreator  Inputs=5
  Gain : Gain  Gain=YBT_Par.Finger_B.Motor.K/YBT_Par.Finger_B.Motor.gr
  PS-Simulink Converter : nesl_utility/PS-Simulink Converter  PhysicalDomain=network_engine_domain  SubClassName=ps_output  LeftPortType=input  RightPortType=output  PseudoPeriodic=off  Frequencies=[]  VectorFormat=1-D array  Unit=mm  AffineConversion=off
  PS-Simulink Converter1 : nesl_utility/PS-Simulink Converter  PhysicalDomain=network_engine_domain  SubClassName=ps_output  LeftPortType=input  RightPortType=output  PseudoPeriodic=off  Frequencies=[]  VectorFormat=1-D array  Unit=1  AffineConversion=off
  PS-Simulink Converter7 : nesl_utility/PS-Simulink Converter  PhysicalDomain=network_engine_domain  SubClassName=ps_output  LeftPortType=input  RightPortType=output  PseudoPeriodic=off  Frequencies=[]  VectorFormat=1-D array  Unit=mm/s  AffineConversion=off
  PS-Simulink Converter8 : nesl_utility/PS-Simulink Converter  PhysicalDomain=network_engine_domain  SubClassName=ps_output  LeftPortType=input  RightPortType=output  PseudoPeriodic=off  Frequencies=[]  VectorFormat=1-D array  Unit=N  AffineConversion=off
  p : PMIOPort  Side=Left
  v : PMIOPort  Port=2  Side=Left
  f : PMIOPort  Port=3  Side=Left
  fc : PMIOPort  Port=4  Side=Left
  b : Outport  VectorParamsAs1DForOutWhenUnconnected=off
  wires:
  Bus Creator/1 -> b/1  "b"
  PS-Simulink Converter7/1 -> Bus Creator/2  "v"
  PS-Simulink Converter/1 -> Bus Creator/1  "p"
  PS-Simulink Converter8/1 -> Gain/1, Bus Creator/3  "f"
  Abs/1 -> Bus Creator/4  "i"
  Gain/1 -> Abs/1
  PS-Simulink Converter1/1 -> Bus Creator/5  "fc"
  connections:
  PS-Simulink Converter8/LConn1 -- f/RConn1
  PS-Simulink Converter7/LConn1 -- v/RConn1
  PS-Simulink Converter/LConn1 -- p/RConn1
  PS-Simulink Converter1/LConn1 -- fc/RConn1

== system youBot_Arm/Arm/Actuation/Motor/Bicep ==
  C : Inport
  Ideal : Subsystem  VariantControl=Ideal
      mask Display: image('youBot_Arm_Actuation_Motor_Ideal_IMAGE.jpg');
  Motor : Subsystem  VariantControl=Motor
      mask Display: image('youBot_Arm_Actuation_Motor_Motor_IMAGE.jpg');
  Test Motor : Subsystem  VariantControl=Test_Motor
  B : PMIOPort  Side=Left
  F : PMIOPort  Port=2  Side=Right
  + : PMIOPort  Port=3  Side=Left
  - : PMIOPort  Port=4  Side=Right
  m : Outport  VectorParamsAs1DForOutWhenUnconnected=off

== system youBot_Arm/Arm/Actuation/Motor/Finger A ==
  C : Inport
  Current Source : fl_lib/Electrical/Electrical Sources/Controlled Current Source
  Meas a : Subsystem
      mask Display: disp('m')
  PS Abs : MyMath_lib/PS Abs
      settings: InternalSimscapePortConfiguration="{\"Bottom\":[],\"Left\":[{\"id\":\"I\",\"label\":\"\",\"type\":\"input\"}],\"Right\":[{\"id\":\"O\",\"label\":\"\",\"type\":\"output\"}],\"Top\":[]}"
  PS Motor Const : fl_lib/Physical Signals/Functions/PS Gain  gain=YBT_Par.Finger_A.Motor.K/YBT_Par.Finger_A.Motor.gr s^2 / (kg*m)
  PrismaticFingerA : sm_lib/Joints/Prismatic Joint  JointMode=Normal  CompositeWrenchDir=FollowerOnBase  CompositeWrenchFrame=BaseFrame  SenseConstraintForce=on  SenseConstraintTorque=off  SenseTotalForce=off  SenseTotalTorque=off  PositionTargetSpecify=on  PositionTargetPriority=Low  PositionTargetValue=smiData.PrismaticJoint(2).Pz.Pos  PositionTargetValueUnits=m  VelocityTargetSpecify=off  VelocityTargetPriority=High  VelocityTargetValue=0  VelocityTargetValueUnits=m/s  EquilibriumPosition=0  EquilibriumPositionUnits=m  SpringStiffness=0  SpringStiffnessUnits=N/m  DampingCoefficient=YBT_Par.Finger_A.Motor.friction  DampingCoefficientUnits=N/(m/s)  LowerLimitSpecify=off  LowerLimitBound=-1  LowerLimitBoundUnits=m  LowerLimitStiffness=1e6  LowerLimitStiffnessUnits=N/m  LowerLimitDamping=1e3  LowerLimitDampingUnits=N/(m/s)  LowerLimitTransitionRegionWidth=1e-4  LowerLimitTransitionRegionWidthUnits=m  UpperLimitSpecify=off  UpperLimitBound=1  UpperLimitBoundUnits=m  UpperLimitStiffness=1e6  UpperLimitStiffnessUnits=N/m  UpperLimitDamping=1e3  UpperLimitDampingUnits=N/(m/s)  UpperLimitTransitionRegionWidth=1e-4  UpperLimitTransitionRegionWidthUnits=m  TorqueActuationMode=ComputedTorque  MotionActuationMode=InputMotion  SensePosition=on  SenseVelocity=on  SenseAcceleration=off  SenseTorqueForce=on  SenseLowerLimitTorqueForce=off  SenseUpperLimitTorqueForce=off
  Resistor : fl_lib/Electrical/Electrical Elements/Resistor  R=YBT_Par.Finger_A.Motor.R Ohm  i_specify=off  i_priority=None  i=0 A  i_nominal_specify=off  i_nominal_value=1  i_nominal_unit=A  v_specify=off  v_priority=None  v=0 V  v_nominal_specify=off  v_nominal_value=1  v_nominal_unit=V
  Simulink-PS Converter3 : nesl_utility/Simulink-PS Converter  Tag=CustomStyle  PhysicalDomain=network_engine_domain  SubClassName=ps_input  LeftPortType=input  RightPortType=output  PseudoPeriodic=off  Frequencies=[]  NoiseDistribution=none  NoiseParameters=[]  Unit=mm  AffineConversion=off  FilteringAndDerivatives=filter  SimscapeFilterOrder=2  InputFilterTimeConstant=0.005  UdotUserProvided=1
  B : PMIOPort  Side=Left
  F : PMIOPort  Port=2  Side=Right
  + : PMIOPort  Port=3  Side=Left
  - : PMIOPort  Port=4  Side=Right
  m : Outport  VectorParamsAs1DForOutWhenUnconnected=off
  wires:
  C/1 -> Simulink-PS Converter3/1
  Meas a/1(m) -> m/1
  connections:
  PrismaticFingerA/LConn1 -- B/RConn1
  PrismaticFingerA/RConn1 -- F/RConn1
  Current Source/RConn2 -- +/RConn1
  PrismaticFingerA/RConn2 -- Meas a/LConn1
  PrismaticFingerA/RConn3 -- Meas a/LConn2
  PrismaticFingerA/RConn4 -- PS Motor Const/LConn1 -- Meas a/LConn3
  PrismaticFingerA/LConn2 -- Simulink-PS Converter3/RConn1
  PS Abs/RConn1 -- Meas a/LConn5 -- Current Source/RConn1
  PS Motor Const/RConn1 -- PS Abs/LConn1
  Resistor/LConn1 -- Current Source/LConn1
  -/RConn1 -- Resistor/RConn1
  PrismaticFingerA/RConn5 -- Meas a/LConn4

== system youBot_Arm/Arm/Actuation/Motor/Finger B ==
  C : Inport
  Current Source : fl_lib/Electrical/Electrical Sources/Controlled Current Source
  Meas b : Subsystem
      mask Display: disp('m')
  PS Abs : MyMath_lib/PS Abs
      settings: InternalSimscapePortConfiguration="{\"Bottom\":[],\"Left\":[{\"id\":\"I\",\"label\":\"\",\"type\":\"input\"}],\"Right\":[{\"id\":\"O\",\"label\":\"\",\"type\":\"output\"}],\"Top\":[]}"
  PS Motor Const : fl_lib/Physical Signals/Functions/PS Gain  gain=YBT_Par.Finger_B.Motor.K/YBT_Par.Finger_B.Motor.gr s^2 / (kg*m)
  PrismaticFingerB : sm_lib/Joints/Prismatic Joint  JointMode=Normal  CompositeWrenchDir=FollowerOnBase  CompositeWrenchFrame=BaseFrame  SenseConstraintForce=on  SenseConstraintTorque=off  SenseTotalForce=off  SenseTotalTorque=off  PositionTargetSpecify=on  PositionTargetPriority=Low  PositionTargetValue=smiData.PrismaticJoint(1).Pz.Pos  PositionTargetValueUnits=m  VelocityTargetSpecify=off  VelocityTargetPriority=High  VelocityTargetValue=0  VelocityTargetValueUnits=m/s  EquilibriumPosition=0  EquilibriumPositionUnits=m  SpringStiffness=0  SpringStiffnessUnits=N/m  DampingCoefficient=YBT_Par.Finger_B.Motor.friction  DampingCoefficientUnits=N/(m/s)  LowerLimitSpecify=off  LowerLimitBound=-1  LowerLimitBoundUnits=m  LowerLimitStiffness=1e6  LowerLimitStiffnessUnits=N/m  LowerLimitDamping=1e3  LowerLimitDampingUnits=N/(m/s)  LowerLimitTransitionRegionWidth=1e-4  LowerLimitTransitionRegionWidthUnits=m  UpperLimitSpecify=off  UpperLimitBound=1  UpperLimitBoundUnits=m  UpperLimitStiffness=1e6  UpperLimitStiffnessUnits=N/m  UpperLimitDamping=1e3  UpperLimitDampingUnits=N/(m/s)  UpperLimitTransitionRegionWidth=1e-4  UpperLimitTransitionRegionWidthUnits=m  TorqueActuationMode=ComputedTorque  MotionActuationMode=InputMotion  SensePosition=on  SenseVelocity=on  SenseAcceleration=off  SenseTorqueForce=on  SenseLowerLimitTorqueForce=off  SenseUpperLimitTorqueForce=off
  Resistor : fl_lib/Electrical/Electrical Elements/Resistor  R=YBT_Par.Finger_B.Motor.R Ohm  i_specify=off  i_priority=None  i=0 A  i_nominal_specify=off  i_nominal_value=1  i_nominal_unit=A  v_specify=off  v_priority=None  v=0 V  v_nominal_specify=off  v_nominal_value=1  v_nominal_unit=V
  Simulink-PS Converter6 : nesl_utility/Simulink-PS Converter  Tag=CustomStyle  PhysicalDomain=network_engine_domain  SubClassName=ps_input  LeftPortType=input  RightPortType=output  PseudoPeriodic=off  Frequencies=[]  NoiseDistribution=none  NoiseParameters=[]  Unit=mm  AffineConversion=off  FilteringAndDerivatives=filter  SimscapeFilterOrder=2  InputFilterTimeConstant=0.005  UdotUserProvided=1
  B : PMIOPort  Side=Left
  F : PMIOPort  Port=2  Side=Right
  + : PMIOPort  Port=3  Side=Left
  - : PMIOPort  Port=4  Side=Right
  m : Outport  VectorParamsAs1DForOutWhenUnconnected=off
  wires:
  C/1 -> Simulink-PS Converter6/1
  Meas b/1(m) -> m/1
  connections:
  PrismaticFingerB/RConn1 -- F/RConn1
  PrismaticFingerB/LConn1 -- B/RConn1
  Current Source/RConn2 -- +/RConn1
  PrismaticFingerB/RConn4 -- PS Motor Const/LConn1 -- Meas b/LConn3
  PrismaticFingerB/RConn3 -- Meas b/LConn2
  PrismaticFingerB/RConn2 -- Meas b/LConn1
  PrismaticFingerB/LConn2 -- Simulink-PS Converter6/RConn1
  PS Abs/RConn1 -- Meas b/LConn5 -- Current Source/RConn1
  -/RConn1 -- Resistor/RConn1
  PS Motor Const/RConn1 -- PS Abs/LConn1
  Resistor/LConn1 -- Current Source/LConn1
  PrismaticFingerB/RConn5 -- Meas b/LConn4

== system youBot_Arm/Arm/Actuation/Motor/Forearm ==
  C : Inport
  Ideal : Subsystem  Tag=PublishSubsystem  VariantControl=Ideal
      mask Display: image('youBot_Arm_Actuation_Motor_Ideal_IMAGE.jpg');
  Motor : Subsystem  Tag=PublishSubsystem  VariantControl=Motor
      mask Display: image('youBot_Arm_Actuation_Motor_Motor_IMAGE.jpg');
  B : PMIOPort  Side=Left
  F : PMIOPort  Port=2  Side=Right
  + : PMIOPort  Port=3  Side=Left
  - : PMIOPort  Port=4  Side=Right
  m : Outport  VectorParamsAs1DForOutWhenUnconnected=off

== system youBot_Arm/Arm/Actuation/Motor/Gripper ==
  C : Inport
  Ideal : Subsystem  VariantControl=Ideal
      mask Display: image('youBot_Arm_Actuation_Motor_Ideal_IMAGE.jpg');
  Motor : Subsystem  VariantControl=Motor
      mask Display: image('youBot_Arm_Actuation_Motor_Motor_IMAGE.jpg');
  B : PMIOPort  Side=Left
  F : PMIOPort  Port=2  Side=Right
  + : PMIOPort  Port=3  Side=Left
  - : PMIOPort  Port=4  Side=Right
  m : Outport  VectorParamsAs1DForOutWhenUnconnected=off

== system youBot_Arm/Arm/Actuation/Motor/Pivot ==
  C : Inport
  Ideal : Subsystem  VariantControl=Ideal
      mask Display: image('youBot_Arm_Actuation_Motor_Ideal_IMAGE.jpg');
  Motor : Subsystem  VariantControl=Motor
      mask Display: image('youBot_Arm_Actuation_Motor_Motor_IMAGE.jpg');
  Test Motor : Subsystem  VariantControl=Test_Motor
  B : PMIOPort  Side=Left
  F : PMIOPort  Port=2  Side=Right
  + : PMIOPort  Port=3  Side=Left
  - : PMIOPort  Port=4  Side=Right
  m : Outport  VectorParamsAs1DForOutWhenUnconnected=off

== system youBot_Arm/Arm/Actuation/Motor/Wrist ==
  C : Inport
  Ideal : Subsystem  VariantControl=Ideal
      mask Display: image('youBot_Arm_Actuation_Motor_Ideal_IMAGE.jpg');
  Motor : Subsystem  VariantControl=Motor
      mask Display: image('youBot_Arm_Actuation_Motor_Motor_IMAGE.jpg');
  B : PMIOPort  Side=Left
  F : PMIOPort  Port=2  Side=Right
  + : PMIOPort  Port=3  Side=Left
  - : PMIOPort  Port=4  Side=Right
  m : Outport  VectorParamsAs1DForOutWhenUnconnected=off

== system youBot_Arm/Arm/Environment/Conveyors/Belt In ==
  On : Inport
  Belt : Subsystem  Tag=CustomStyle  mask(Conveyor Belt, 5 Rollers){belt_l=YBT_Par.BeltIn.length, belt_d=YBT_Par.BeltIn.depth, belt_w=YBT_Par.BeltIn.width, roller_clr=YBT_Par.BeltIn.Roller.color, ctrrefnorm_popup=+Z}
      mask prompts: belt_l "Conveyor Length (m)"; belt_d "Conveyor Depth (m)"; belt_w "Conveyor Width (m)"; roller_clr "Roller Color (rgb)"; ctrrefnorm_popup "Center Reference Frame, Normal Axis"
      mask help: Models a conveyor belt. Input signal is belt speed which only affects roller rotational speed in animation.
      mask init:
      | temp_curblk = gcb;
      | if strcmp(get_param(temp_curblk,'ctrrefnorm_popup'),'+Z')
      |     set_param([temp_curblk '/Transform Contact Ref'],'RotationSequenceAngles','[-90 0 0]');
      | elseif strcmp(get_param(temp_curblk,'ctrrefnorm_popup'),'+X')
      |     set_param([temp_curblk '/Transform Contact Ref'],'RotationSequenceAngles','[0 0 90]');
      | end
      | clear temp_curblk
      mask TypeOptions ctrrefnorm_popup: +Z | +X
      mask Display: image('youBot_Arm_Belt_IMAGE.jpg');
  Belt Speed : Gain  Gain=0.1
  Box to Belt In Force : Contact_Forces_Lib/3D/Composite Forces/Face to Belt Faces Force  PlaB_x=YBT_Par.BeltIn.length  PlaB_y=YBT_Par.BeltIn.width  PlaB_z=YBT_Par.BeltIn.depth/2  FacF_x=YBT_Par.Cube.d  FacF_y=YBT_Par.Cube.d  FacF_z=YBT_Par.Cube.d/2  FacF_rSph=YBT_Par.Cube.Con.rSph  force_law_pla2pla=Linear  k_contact_pla2pla=1e3  b_contact_pla2pla=1e2  pen_full_damp_F_pla2pla=1e-4  pen_exponent_pla2pla=1  friction_law_pla2pla=Stick-Slip Continuous  mu_kinetic_pla2pla=0.5  mu_static_pla2pla=0.7  v_thr_pla2pla=0.001  vis_on_pla2pla=off  vis_opc_en_box2box=0  vis_len_plaLz=0.0005  vis_clr=[0.9 0.2 0.2]  vis_opc=0.7
      settings: SourceProductName=Simscape Multibody Contact Forces Library
  Bus Creator : BusCreator  Inputs=2
  Create Bus : Subsystem
  Detect Box : Subsystem  mask{box_weight=YBT_Par.Payload.max_m, dur_presence=YBT_Par.BeltIn.Control.Delay_on}
      mask prompts: box_weight "Box Weight (kg)"; dur_presence "Duration for Presence (s)"
  Light Curtain : Subsystem
      mask Display: image('youBot_Arm_Belt_Light_Curtain_IMAGE.jpg');
  Normal Force : Subsystem
  Transform Light Curtain : sm_lib/Frames and Transforms/Rigid Transform  RotationMethod=None  FollAlignAxisA=+X  BaseAlignAxisA=+Y  FollAlignAxisB=+Y  BaseAlignAxisB=+Z  RotationStandardAxis=+Y  RotationAngle=0  RotationAngleUnits=deg  RotationArbitraryAxis=[0 0 1]  RotationSequenceAxes=FollowerAxes  RotationSequence=XYX  RotationSequenceAngles=[0 0 0]  RotationSequenceAnglesUnits=deg  RotationMatrix=[1 0 0; 0 1 0; 0 0 1]  Quaternion=[1 0 0 0]  TranslationMethod=Cartesian  TranslationCartesianOffset=YBT_Par.BeltIn.Sensor.offset  TranslationCartesianOffsetUnits=m  TranslationStandardAxis=+Y  TranslationStandardOffset=0  TranslationStandardOffsetUnits=m  TranslationROffset=0  TranslationROffsetUnits=m  TranslationThetaOffset=0  TranslationThetaOffsetUnits=deg  TranslationZOffset=0  TranslationZOffsetUnits=m
  Box : PMIOPort  Side=Right
  Floor : PMIOPort  Port=2  Side=Left
  Sensors : Outport  VectorParamsAs1DForOutWhenUnconnected=off
  wires:
  Box to Belt In Force/1 -> Normal Force/1(bus)
  Create Bus/1(bus) -> Box to Belt In Force/1
  Light Curtain/1(p) -> Bus Creator/2  "LC"
  On/1 -> Belt Speed/1
  Belt Speed/1 -> Belt/1(Spd), Create Bus/1(vx)  "vx"
  Normal Force/1(sum) -> Detect Box/1(Fn)
  Detect Box/1(On) -> Bus Creator/1  "Box"
  Bus Creator/1 -> Sensors/1  "BeltIn"
  connections:
  Box/RConn1 -- Box to Belt In Force/LConn1 -- Light Curtain/RConn1
  Box to Belt In Force/RConn1 -- Belt/RConn1 -- Transform Light Curtain/LConn1 -- Floor/RConn1
  Light Curtain/LConn1 -- Transform Light Curtain/RConn1

== system youBot_Arm/Arm/Environment/Conveyors/Belt Out ==
  On : Inport
  Belt : Subsystem  Tag=CustomStyle  mask(Conveyor Belt, 5 Rollers){belt_l=YBT_Par.BeltOut.length, belt_d=YBT_Par.BeltOut.depth, belt_w=YBT_Par.BeltOut.width, roller_clr=YBT_Par.BeltOut.Roller.color, ctrrefnorm_popup=+Z}
      mask prompts: belt_l "Conveyor Length (m)"; belt_d "Conveyor Depth (m)"; belt_w "Conveyor Width (m)"; roller_clr "Roller Color (rgb)"; ctrrefnorm_popup "Center Reference Frame, Normal Axis"
      mask help: Models a conveyor belt. Input signal is belt speed which only affects roller rotational speed in animation.
      mask init: same as youBot_Arm/Arm/Environment/Conveyors/Belt In/Belt
      mask TypeOptions ctrrefnorm_popup: +Z | +X
      mask Display: image('youBot_Arm_Belt_IMAGE.jpg');
  Belt Speed : Gain  Gain=0.1
  Box to Belt In Force : Contact_Forces_Lib/3D/Composite Forces/Face to Belt Faces Force  PlaB_x=YBT_Par.BeltIn.length  PlaB_y=YBT_Par.BeltIn.width  PlaB_z=YBT_Par.BeltIn.depth/2  FacF_x=YBT_Par.Cube.d  FacF_y=YBT_Par.Cube.d  FacF_z=-YBT_Par.Cube.d/2  FacF_rSph=YBT_Par.Cube.Con.rSph  force_law_pla2pla=Linear  k_contact_pla2pla=1e3  b_contact_pla2pla=1e2  pen_full_damp_F_pla2pla=1e-4  pen_exponent_pla2pla=1  friction_law_pla2pla=Stick-Slip Continuous  mu_kinetic_pla2pla=0.5  mu_static_pla2pla=0.7  v_thr_pla2pla=0.001  vis_on_pla2pla=off  vis_opc_en_box2box=0  vis_len_plaLz=0.0005  vis_clr=[0.9 0.2 0.2]  vis_opc=0.7
      settings: SourceProductName=Simscape Multibody Contact Forces Library
  Bus Creator : BusCreator  Inputs=2
  Create Bus : Subsystem
  Detect Box : Subsystem  mask{box_weight=YBT_Par.Payload.max_m, dur_presence=YBT_Par.BeltOut.Control.Delay_on}
      mask prompts: box_weight "Box Weight (kg)"; dur_presence "Duration for Presence (s)"
  Light Curtain : Subsystem
      mask Display: image('youBot_Arm_Belt_Light_Curtain_IMAGE.jpg');
  Normal Force : Subsystem
  Transform Light Curtain : sm_lib/Frames and Transforms/Rigid Transform  RotationMethod=None  FollAlignAxisA=+X  BaseAlignAxisA=+Y  FollAlignAxisB=+Y  BaseAlignAxisB=+Z  RotationStandardAxis=+Y  RotationAngle=0  RotationAngleUnits=deg  RotationArbitraryAxis=[0 0 1]  RotationSequenceAxes=FollowerAxes  RotationSequence=XYX  RotationSequenceAngles=[0 0 0]  RotationSequenceAnglesUnits=deg  RotationMatrix=[1 0 0; 0 1 0; 0 0 1]  Quaternion=[1 0 0 0]  TranslationMethod=Cartesian  TranslationCartesianOffset=YBT_Par.BeltOut.Sensor.offset  TranslationCartesianOffsetUnits=m  TranslationStandardAxis=+Y  TranslationStandardOffset=0  TranslationStandardOffsetUnits=m  TranslationROffset=0  TranslationROffsetUnits=m  TranslationThetaOffset=0  TranslationThetaOffsetUnits=deg  TranslationZOffset=0  TranslationZOffsetUnits=m
  Box : PMIOPort  Side=Right
  Floor : PMIOPort  Port=2  Side=Left
  Sensors : Outport  VectorParamsAs1DForOutWhenUnconnected=off
  wires:
  Belt Speed/1 -> Create Bus/1(vx), Belt/1(Spd)  "vx"
  On/1 -> Belt Speed/1
  Light Curtain/1(p) -> Bus Creator/2  "LC"
  Create Bus/1(bus) -> Box to Belt In Force/1
  Box to Belt In Force/1 -> Normal Force/1(bus)
  Normal Force/1(sum) -> Detect Box/1(Fn)
  Detect Box/1(On) -> Bus Creator/1  "Box"
  Bus Creator/1 -> Sensors/1  "BeltOut"
  connections:
  Light Curtain/LConn1 -- Transform Light Curtain/RConn1
  Box to Belt In Force/RConn1 -- Floor/RConn1 -- Transform Light Curtain/LConn1 -- Belt/RConn1
  Light Curtain/RConn1 -- Box to Belt In Force/LConn1 -- Box/RConn1

== system youBot_Arm/Arm/Environment/Gripper Force/Damper ==
  Gripper Force : Subsystem  Tag=PublishSubsystem  mask(Gripper Fingers to Load Force){cube_z=YBT_Par.Cube.d, contact_b=YBT_Par.Finger.Con.damper, lpf_const_gripper_force=0.05, popup_relvel=Relative velocity wrt. gripper housing}
      mask prompts: cube_z "Cube Length (m)"; contact_b "Damping Coefficient"; lpf_const_gripper_force "Low pass filter constant (s)"; popup_relvel "Load-gripper relative velocity along finger normal calculation:"
      mask help:
      | Models the force between the gripper fingers and the load as a controlled damper.  A very stiff 6-degree of freedom damping force becomes active when the load is between the fingers and the gripper fingers are closed enough to grasp the load.  This abstract method makes many assumptions about the interaction between the gripper and the load.
      |
      | Two options are provided to measure the velocity of the load normal to the gripper fingers.
      |
      | 1. Difference of relative velocity wrt. each finger
      | 2. Relative velocity wrt. gripper housing
      mask init:
      | temp_popup_relvel = get_param(gcb,'popup_relvel');
      | 
      | if (strncmpi(temp_popup_relvel,'Differ',6))
      |     set_param([gcb '/Relative vz'],'OverrideUsingVariant','Fingers');
      | else
      |     set_param([gcb '/Relative vz'],'OverrideUsingVariant','Housing');
      | end
      | 
      | clear temp_popup_relvel
      mask TypeOptions popup_relvel: Difference of relative velocities wrt. each finger | Relative velocity wrt. gripper housing
      mask DialogControl Container6 Prompt: Geometry
      mask DialogControl Container7 Prompt: Force
  Fa : PMIOPort  Side=Right
  Bfa : PMIOPort  Port=2  Side=Left
  E : PMIOPort  Port=3  Side=Right
  Fb : PMIOPort  Port=4  Side=Right
  Bfb : PMIOPort  Port=5  Side=Left
  connections:
  Gripper Force/RConn3 -- Fb/RConn1
  Gripper Force/RConn1 -- Fa/RConn1
  Gripper Force/LConn1 -- Bfb/RConn1
  E/RConn1 -- Gripper Force/RConn2

== system youBot_Arm/Arm/Environment/Gripper Force/Payload ==
  Load : sm_lib/Body Elements/Brick Solid  BrickDimensions=[1 1 1]*YBT_Par.Payload.Cube.d  BrickDimensionsUnits=m  ExportEntireGeometry=off  InertiaType=CalculateFromGeometry  BasedOnType=Density  Density=YBT_Par.Payload.Cube.rho  DensityUnits=kg/m^3  Mass=1  MassUnits=kg  CenterOfMass=[0 0 0]  CenterOfMassUnits=m  MomentsOfInertia=[1 1 1]  MomentsOfInertiaUnits=kg*m^2  ProductsOfInertia=[1 1 1]  ProductsOfInertiaUnits=kg*m^2  GraphicType=FromGeometry  MarkerShape=Sphere  MarkerSize=10  GraphicVisPropType=SimpleVisualProperties  GraphicDiffuseColor=[0.6 0.8 1.0]  GraphicOpacity=1  GraphicSpecularColor=[0.5 0.5 0.5 1.0]  GraphicAmbientColor=[0.15 0.15 0.15 1.0]  GraphicEmissiveColor=[0.0 0.0 0.0 1.0]  GraphicShininess=75  DoExposeReferenceFrame=on  SerializedFrames=<Frames/>
  Marks : Subsystem
  Rigid Transform : sm_lib/Frames and Transforms/Rigid Transform  RotationMethod=StandardAxis  FollAlignAxisA=+X  BaseAlignAxisA=+Y  FollAlignAxisB=+Y  BaseAlignAxisB=+Z  RotationStandardAxis=+Y  RotationAngle=90  RotationAngleUnits=deg  RotationArbitraryAxis=[0 0 1]  RotationSequenceAxes=FollowerAxes  RotationSequence=XYX  RotationSequenceAngles=[0 0 0]  RotationSequenceAnglesUnits=deg  RotationMatrix=[1 0 0; 0 1 0; 0 0 1]  Quaternion=[1 0 0 0]  TranslationMethod=None  TranslationCartesianOffset=[0 0 0]  TranslationCartesianOffsetUnits=m  TranslationStandardAxis=+Z  TranslationStandardOffset=0  TranslationStandardOffsetUnits=m  TranslationROffset=0  TranslationROffsetUnits=m  TranslationThetaOffset=0  TranslationThetaOffsetUnits=deg  TranslationZOffset=0  TranslationZOffsetUnits=m
  Fa : PMIOPort  Side=Right
  Bfa : PMIOPort  Port=2  Side=Left
  E : PMIOPort  Port=3  Side=Right
  Fb : PMIOPort  Port=4  Side=Right
  Bfb : PMIOPort  Port=5  Side=Left
  connections:
  Rigid Transform/LConn1 -- E/RConn1
  Rigid Transform/RConn1 -- Marks/LConn1 -- Load/RConn1

== system youBot_Arm/Arm/Environment/Gripper Force/Penalty ==
  Plane to Face Force Fa : Contact_Forces_Lib/3D/Composite Forces/Face to Plane Force  PlaB_x=YBT_Par.Cube.d  PlaB_y=YBT_Par.Cube.d  PlaB_z=YBT_Par.Cube.d/2  FacF_x=YBT_Par.Finger.Con.x  FacF_y=YBT_Par.Finger.Con.y  FacF_z=YBT_Par.Finger.Con.z  FacF_rSph=YBT_Par.Finger.Con.rSph  force_law_pla2pla=Linear  k_contact_pla2pla=YBT_Par.Finger.Con.k  b_contact_pla2pla=YBT_Par.Finger.Con.b  pen_full_damp_F_pla2pla=1e-4  pen_exponent_pla2pla=1  friction_law_pla2pla=Stick-Slip Continuous  mu_kinetic_pla2pla=YBT_Par.Finger.Con.muk  mu_static_pla2pla=YBT_Par.Finger.Con.mus  v_thr_pla2pla=YBT_Par.Finger.Con.vth  vis_on_pla2pla=off  vis_opc_en_box2box=0  vis_len_plaLz=0.0005  vis_clr=[0.9 0.2 0.2]  vis_opc=0.7
      settings: SourceProductName=Simscape Multibody Contact Forces Library
  Plane to Face Force Fb : Contact_Forces_Lib/3D/Composite Forces/Face to Plane Force  PlaB_x=YBT_Par.Cube.d  PlaB_y=YBT_Par.Cube.d  PlaB_z=YBT_Par.Cube.d/2  FacF_x=YBT_Par.Finger.Con.x  FacF_y=YBT_Par.Finger.Con.y  FacF_z=YBT_Par.Finger.Con.z  FacF_rSph=YBT_Par.Finger.Con.rSph  force_law_pla2pla=Linear  k_contact_pla2pla=YBT_Par.Finger.Con.k  b_contact_pla2pla=YBT_Par.Finger.Con.b  pen_full_damp_F_pla2pla=1e-4  pen_exponent_pla2pla=1  friction_law_pla2pla=Stick-Slip Continuous  mu_kinetic_pla2pla=0.5  mu_static_pla2pla=0.7  v_thr_pla2pla=0.001  vis_on_pla2pla=off  vis_opc_en_box2box=0  vis_len_plaLz=0.0005  vis_clr=[0.9 0.2 0.2]  vis_opc=0.7
      settings: SourceProductName=Simscape Multibody Contact Forces Library
  Sc2 : Subsystem
  Terminator : Terminator
  Fa : PMIOPort  Side=Right
  Bfa : PMIOPort  Port=2  Side=Left
  E : PMIOPort  Port=3  Side=Right
  Fb : PMIOPort  Port=4  Side=Right
  Bfb : PMIOPort  Port=5  Side=Left
  wires:
  Plane to Face Force Fa/1 -> Sc2/1(In1)
  Plane to Face Force Fb/1 -> Terminator/1
  connections:
  Plane to Face Force Fb/RConn1 -- Bfb/RConn1
  Plane to Face Force Fa/RConn1 -- Bfa/RConn1
  Plane to Face Force Fa/LConn1 -- Fa/RConn1
  Plane to Face Force Fb/LConn1 -- Fb/RConn1
